simulink model "Inverter_pq_comp_sat"  (R2023b)
settings: Solver=FixedStepDiscrete  StartTime=0.0  StopTime=0.04  RelTol=1e-3  EnableMultiTasking=on
InitFcn:
  | %% Definition of the parameters
  | 
  | Parameter_Definition
  | 
  | %% Damping
  | 
  | Rd = 3.9;
  | 
  | %% PRes Gains Calculation
  | 
  | % Definicao das grandezas
  | w_cl = 1j*2*pi*1200;  % Phase Crossing Frequency
  | no   = 1;           % Integral Resonant Constant
  | A    = 1;             % Carrier Amplitude
  | 
  | % Kp calculation
  | a0 = 1;
  | a1 = Rd*Cf;
  | b0 = 0;
  | b1 = Lf+Lg;
  | b2 = Rd*Lf*Cf+Rd*Lg*Cf;
  | b3 = Lf*Lg*Cf;
  | 
  | G_lcl = (a1*w_cl+a0)/(b3*w_cl^3+b2*w_cl^2+b1*w_cl+b0);
  | % G_lcl = 1/((Lf+Lg)*w_cl+Rf);
  | 
  | G_PWM = (1/A)*(1-w_cl*Ts/4)/(1+w_cl*Ts/4);
  | 
  | G_wc  = (Vdc/2)*(1/I_base)*G_lcl*G_PWM;
  | 
  | G_wc_abs = abs(G_wc);
  | 
  | Kp = 0.8/G_wc_abs;
  | 
  | % Discretized Controller Gains
  | ressonance_list = [1,5,7];
  | 
  | n_res = length(ressonance_list);
  | a = zeros(2,n_res);
  | b = zeros(2,n_res);
  | Ki_res = zeros(1,n_res);
  | 
  | % for i = 1:n_res
  | %   k = ressonance_list(i);
  | %   Ki_res(i) = (2.2*Kp)/(no*T_gr);
  | %   a(i) = (2*Ki_res(i)*Ts)/(4+((k*w_gr)^2)*Ts^2);
  | %   b(i) = (-8+2*((k*w_gr)^2)*Ts^2)/(4+((k*w_gr)^2)*Ts^2);
  | % end
  | 
  | % wc is the cutoff frequency/damping factor in rad/s
  | wc = 5;
  | 
  | for i = 1:n_res
  |   k = ressonance_list(i);
  |   wk = k * w_gr; % Resonant frequency for this harmonic
  | 
  |   Ki_res(i) = (2.2*Kp)/(no*T_gr);
  | 
  |   % 1. Calculate the common denominator
  |   den = 4 + 4*wc*Ts + (wk^2)*(Ts^2);
  | 
  |   % 2. Calculate the numerator terms (A coefficients for the input x)
  |   num_A0 = 2 * Ki_res(i) * wc * Ts;
  | 
  |   % 3. Calculate the denominator terms (B coefficients for the output y)
  |   num_B1 = -8 + 2*(wk^2)*(Ts^2);
  |   num_B2 = 4 - 4*wc*Ts + (wk^2)*(Ts^2);
  | 
  |   % 4. Normalize the coefficients
  |   a(1,i) = num_A0 / den;
  |   a(2,i) = -1*num_A0 / den;
  |   b(1,i) = num_B1 / den;
  |   b(2,i) = num_B2 / den;
  | end
values from neighbouring files (symbols this model uses):
  a1_sogi = single(2*(w0_sogi^2-c_sogi^2)/den0_sogi)    [Parameter_Definition.m]
  a2_sogi = single((c_sogi^2                 - k_sogi*w0_sogi*c_sogi                 + w0_sogi^2)/den0_sogi)    [Parameter_Definition.m]
  bD_sogi = single(k_sogi*w0_sogi*c_sogi/den0_sogi)    [Parameter_Definition.m]
  bQ_sogi = single(k_sogi*w0_sogi^2/den0_sogi)    [Parameter_Definition.m]
  Cf = 5e-6    (= 5e-06)    [Parameter_Definition.m]
  I_base = S_base/(sqrt(3)*V_gr)    [Parameter_Definition.m]
  K_i = 1/25    (= 0.04)    [Parameter_Definition.m]
  K_vc = 1/200    (= 0.005)    [Parameter_Definition.m]
  K_vdc = 1/500    (= 0.002)    [Parameter_Definition.m]
  Lf = 1e-3    (= 0.001)    [Parameter_Definition.m]
  Lg = 0.5e-3    (= 0.0005)    [Parameter_Definition.m]
  S_base = S_rated    (= 1000)    [Parameter_Definition.m]
  Ts = 2*(4167)/100e6    (= 8.334e-05)    [Parameter_Definition.m]
  V_base = sqrt(3)*V_gr    [Parameter_Definition.m]
  Vdc = 800    [Parameter_Definition.m]
  Vdc_base = Vdc    (= 800)    [Parameter_Definition.m]
  w_gr = 2*pi*f_gr    (= 376.991118431)    [Parameter_Definition.m]
undefined symbols (not defined in the file or in its folder): Down, gH_LUT, GPTRIP1SEL, gQ_LUT, gV_LUT, lH_vetor, lQ_vetor, lV_vetor, TZ1, Up
libraries: c2802xlib x32, c2837xDlib x4, simulink x1
(part 1 of 3)
settings Model: SimulationMode=external  ExtModeTrigDuration=8  Creator=AugustoMatheusdosSan  LastModifiedBy=engam
settings SolverCC: AutoInsertRateTranBlk=on
settings OptimizationCC: DefaultUnderspecifiedDataType=single  EnhancedBackFolding=on  PassReuseOutputArgsAs=Individual arguments  MaxStackSize=1024  OptimizeBlockOrder=speed  DifferentSizesBufferReuse=on  OptimizationCustomize=off  EfficientTunableParamExpr=on
settings DebuggingCC: ParameterPrecisionLossMsg=none  ParameterTunabilityLossMsg=error
settings HardwareCC: ProdBitPerChar=16  ProdBitPerInt=16  ProdBitPerPointer=32  ProdBitPerSizeT=32  ProdBitPerPtrDiffT=32  ProdLargestAtomicInteger=Integer  ProdLargestAtomicFloat=None  ProdWordSize=16  ProdLongLongMode=on  ProdHWDeviceType=Texas Instruments->C2000  HardwareBoardFeatureSet=SoCBlockset
settings ModelReferenceCC: ModelReferenceNumInstancesAllowed=Single
settings SFSimCC: MATLABDynamicMemAlloc=off
settings RTWCC: Description=Embedded Coder  SystemTargetFile=ert.tlc  HardwareBoard=TI Delfino F2837xD  TemplateMakefile=ert_default_tmf  Toolchain=Texas Instruments Code Composer Studio (C2000)  BuildConfiguration=Faster Runs  CodeProfilingSaveOptions=MetricsOnly
settings CodeAppCC: ForceParamTrailComments=on  IgnoreCustomStorageClasses=off  OperatorAnnotations=on  SimulinkDataObjDesc=on  SFDataObjDesc=on  InsertBlockDesc=on
settings ERTTargetCC: TargetLangStandard=C99 (ISO)  CodeReplacementLibrary=TI C28x  ExtModeTransport=4  ExtModeStaticAlloc=on  ExtModeAutomaticAllocSize=off  ExtModeStaticAllocSize=10000  ExtModeMexFile=ext_xcp  ExtModeIntrfLevel=Level2 - Open  EnableUserReplacementTypes=on

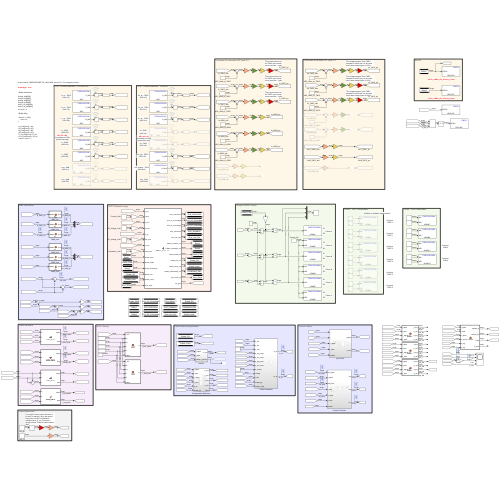
[thumbnail: Simulink's stored preview of the top-level diagram]
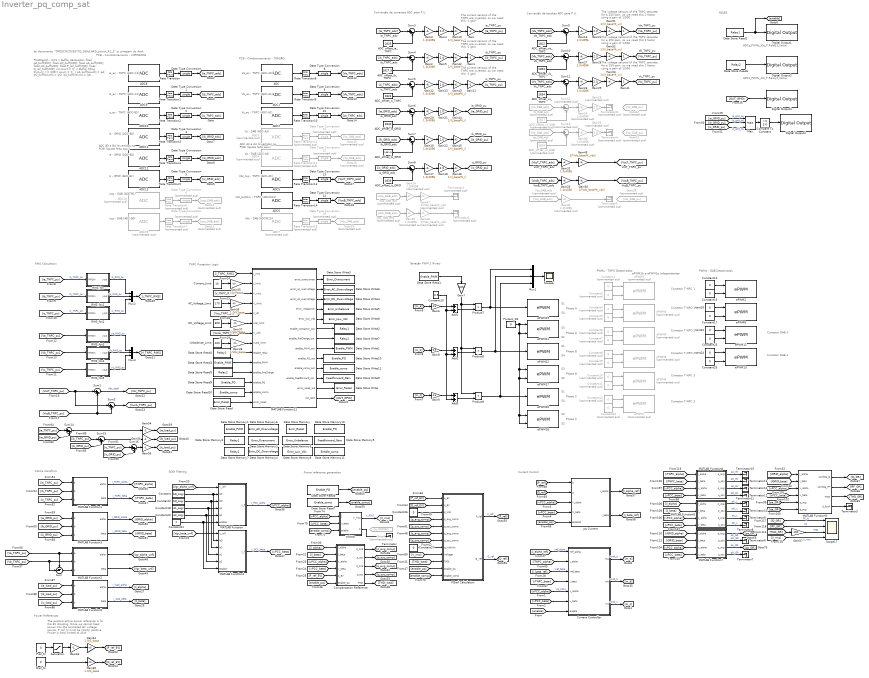
== system Inverter_pq_comp_sat ==
  note: S1
  note: Phase C
  note: The current sensors of the TNPC are inverted, so we need this -1 gain
  note: Conector
      | DAB 3
  note: Conversão de tensões ADC para P.U.
  note: S4
  note: Geração PWM 2 Níveis
  note: Phase C
  note: The current sensors of the TNPC are inverted, so we need this -1 gain
  note: RELÉS
  note: PlotGrapgh - CCS
      |
      | // Buffer declaration
      |
      | float pA_buff[200];
      | float pO_buff[200];
      | float qA_buff[200];
      | float qO_buff[200];
      | float P_ref_buff[200];
      | float Q_ref_buff[200];
      | int count = 0;
      |
      | // Buffer filling
      |
      | if(count >= 200){
      | count = 0;
      | }
      |
      | pA_buff[count] = pA;
      | pO_buff[count] = pO;
      | qA_buff[count] = qA;
      | qO_buff[count] = qO;
      | P_ref_buff[count] = P_ref;
      | Q_ref_buff[count] = Q_ref;
      | count = count + 1;
  note: PWMs - TNPC Desativados
  note: Conversão de correntes ADC para P.U.
  note: ib_ac - TNPC
      | (ADC-C2)
  note: ler documento "TMDSCNCD28377D_180cCARD_pinout_R1_3" p/ pinagem do dock
  note: Vp - DAB
      | (ADC-A4)
  note: PCB - Condicionamento - CORRENTE
  note: Vdc_bottom - TNPC
      | (ADCIN14)
  note: Vb_ac - TNPC
      | (ADC-A1)
  note: Va_ac - TNPC
      | (ADC-A0)
  note: The current sensors of the TNPC are inverted, so we need this -1 gain
  note: Vdc_top - TNPC
      | (ADC-A5)
  note: Vdc - DAB
      | (ADCIN15)
  note: Vs - DAB
      | (ADC-A3)
  note: ic_ac - TNPC
      | (ADC-B5)
  note: ia_ac - TNPC
      | (ADC-C3)
  note: ib - GRID
      | (ADC-B4)
  note: ia - GRID
      | (ADC-B3)
  note: S2
  note: ADCs_PWMs_IOs_P.Relay2_Value
  note: PWMs - DAB Desativados
  note: ADCs_PWMs_IOs_P.Relay1_Value
  note: iccp - DAB
      | (ADC-B1)
  note: iccs - DAB
      | (ADC-B0)
  note: ADC A3 e A4
      | (Invertidos na PCB)
      | (Ajuste feito aqui)
  note: Conector
      | T-NPC 1
  note: ADC B3 e B4
      | (Invertidos na PCB)
      | (Ajuste feito aqui)
  note: Conector
      | T-NPC 2
  note: ePWM1b e ePWM1a independentes
  note: ic - GRID
      | (ADC-B2)
  note: Conector
      | DAB 4
  note: Conector
      | T-NPC 2
  note: Conector
      | T-NPC 3
  note: Phase A
  note: S1
  note: S2
  note: S3
  note: Phase A
  note: PCB - Condicionamento - TENSÃO
  note: S1
  note: Conector
      | T-NPC 1
  note: S4
  note: S2
  note: S3
  note: Phase B
  note: S3
  note: Conector
      | T-NPC 3
  note: Phase B
  note: Vc_ac - TNPC
      | (ADC-A2)
  note: S4
  note: The voltage sensors of the TNPC saturate for a 250 gain, so we need this 2 factor using a gain of 1/500
  note: The voltage sensors of the TNPC saturate for a 250 gain, so we need this 2 factor using a gain of 1/500
  note: The voltage sensors of the TNPC saturate for a 250 gain, so we need this 2 factor using a gain of 1/500
  note: RMS Calculation
  note: The positive active power reference is for the EV charging. Since we cannot feed power into the controlled AC voltage source, P_ref_SI must be strictly positive. Power is hard limited to 4kW
  note: Power References
  note: TNPC Protection Logic
  note: SOGI Filtering
  note: Clarke transform
  note: Current Control
  note: Power reference generation
  AC_Voltage_Limit : Constant  Value=170  OutDataTypeStr=single
  ADC : c2802xlib/ADC  blkParamProc=C2000_Type4  ADCModule=A  samplingMode=Single sample mode  ADCResolution=12-bit (Single-ended input)  useSOC1=SOC0  useSOC2=SOC0_SOC1  SOCAcquisitionWindow=15  SOCTriggerSource=ePWM1_ADCSOCA  SOCInterruptTrigger=No ADCINT  Ts=Ts  dType=single  postInterrupt=off  interruptSel=ADCINT1  ADCINTContinuous=on  endma=off  chdma=1  conv1=ADCINA0  conv2=ADCINA0 and ADCINB0  conv1_Type4=ADCIN0  conv2_Type4=ADCIN0 and ADCIN1
      settings: LibrarySourceBlock=c2837xDlib/ADC
  ADC1 : c2802xlib/ADC  blkParamProc=C2000_Type4  ADCModule=A  samplingMode=Single sample mode  ADCResolution=12-bit (Single-ended input)  useSOC1=SOC1  useSOC2=SOC0_SOC1  SOCAcquisitionWindow=15  SOCTriggerSource=ePWM1_ADCSOCA  SOCInterruptTrigger=No ADCINT  Ts=Ts  dType=single  postInterrupt=off  interruptSel=ADCINT1  ADCINTContinuous=on  endma=off  chdma=1  conv1=ADCINA0  conv2=ADCINA0 and ADCINB0  conv1_Type4=ADCIN1  conv2_Type4=ADCIN0 and ADCIN1
      settings: LibrarySourceBlock=c2837xDlib/ADC
  ADC10 : c2802xlib/ADC  blkParamProc=C2000_Type4  ADCModule=B  samplingMode=Single sample mode  ADCResolution=12-bit (Single-ended input)  useSOC1=SOC10  useSOC2=SOC0_SOC1  SOCAcquisitionWindow=15  SOCTriggerSource=ePWM1_ADCSOCA  SOCInterruptTrigger=No ADCINT  Ts=Ts  dType=single  postInterrupt=off  interruptSel=ADCINT1  ADCINTContinuous=on  endma=off  chdma=1  conv1=ADCINA0  conv2=ADCINA0 and ADCINB0  conv1_Type4=ADCIN5  conv2_Type4=ADCIN0 and ADCIN1
      settings: LibrarySourceBlock=c2837xDlib/ADC
  ADC11 : c2802xlib/ADC  blkParamProc=C2000_Type4  ADCModule=B  samplingMode=Single sample mode  ADCResolution=12-bit (Single-ended input)  useSOC1=SOC11  useSOC2=SOC0_SOC1  SOCAcquisitionWindow=15  SOCTriggerSource=ePWM1_ADCSOCA  SOCInterruptTrigger=No ADCINT  Ts=Ts  dType=double  postInterrupt=off  interruptSel=ADCINT1  ADCINTContinuous=on  endma=off  chdma=1  conv1=ADCINA0  conv2=ADCINA0 and ADCINB0  conv1_Type4=ADCIN4  conv2_Type4=ADCIN0 and ADCIN1
      settings: LibrarySourceBlock=c2837xDlib/ADC
  ADC12 : c2802xlib/ADC  blkParamProc=C2000_Type4  ADCModule=B  samplingMode=Single sample mode  ADCResolution=12-bit (Single-ended input)  useSOC1=SOC12  useSOC2=SOC0_SOC1  SOCAcquisitionWindow=15  SOCTriggerSource=ePWM1_ADCSOCA  SOCInterruptTrigger=No ADCINT  Ts=Ts  dType=double  postInterrupt=off  interruptSel=ADCINT1  ADCINTContinuous=on  endma=off  chdma=1  conv1=ADCINA0  conv2=ADCINA0 and ADCINB0  conv1_Type4=ADCIN3  conv2_Type4=ADCIN0 and ADCIN1
      settings: LibrarySourceBlock=c2837xDlib/ADC
  ADC13 : c2802xlib/ADC  blkParamProc=C2000_Type4  ADCModule=B  samplingMode=Single sample mode  ADCResolution=12-bit (Single-ended input)  useSOC1=SOC13  useSOC2=SOC0_SOC1  SOCAcquisitionWindow=15  SOCTriggerSource=ePWM1_ADCSOCA  SOCInterruptTrigger=No ADCINT  Ts=Ts  dType=double  postInterrupt=off  interruptSel=ADCINT1  ADCINTContinuous=on  endma=off  chdma=1  conv1=ADCINA0  conv2=ADCINA0 and ADCINB0  conv1_Type4=ADCIN2  conv2_Type4=ADCIN0 and ADCIN1
      settings: LibrarySourceBlock=c2837xDlib/ADC
  ADC14 : c2802xlib/ADC  Commented=on  blkParamProc=C2000_Type4  ADCModule=B  samplingMode=Single sample mode  ADCResolution=12-bit (Single-ended input)  useSOC1=SOC14  useSOC2=SOC0_SOC1  SOCAcquisitionWindow=15  SOCTriggerSource=Software  SOCInterruptTrigger=No ADCINT  Ts=Ts  dType=double  postInterrupt=off  interruptSel=ADCINT1  ADCINTContinuous=on  endma=off  chdma=1  conv1=ADCINA0  conv2=ADCINA0 and ADCINB0  conv1_Type4=ADCIN1  conv2_Type4=ADCIN0 and ADCIN1
      settings: LibrarySourceBlock=c2837xDlib/ADC
  ADC15 : c2802xlib/ADC  Commented=on  blkParamProc=C2000_Type4  ADCModule=B  samplingMode=Single sample mode  ADCResolution=12-bit (Single-ended input)  useSOC1=SOC15  useSOC2=SOC0_SOC1  SOCAcquisitionWindow=15  SOCTriggerSource=Software  SOCInterruptTrigger=No ADCINT  Ts=Ts  dType=double  postInterrupt=off  interruptSel=ADCINT1  ADCINTContinuous=on  endma=off  chdma=1  conv1=ADCINA0  conv2=ADCINA0 and ADCINB0  conv1_Type4=ADCIN0  conv2_Type4=ADCIN0 and ADCIN1
      settings: LibrarySourceBlock=c2837xDlib/ADC
  ADC2 : c2802xlib/ADC  blkParamProc=C2000_Type4  ADCModule=A  samplingMode=Single sample mode  ADCResolution=12-bit (Single-ended input)  useSOC1=SOC2  useSOC2=SOC0_SOC1  SOCAcquisitionWindow=15  SOCTriggerSource=ePWM1_ADCSOCA  SOCInterruptTrigger=No ADCINT  Ts=Ts  dType=double  postInterrupt=off  interruptSel=ADCINT1  ADCINTContinuous=on  endma=off  chdma=1  conv1=ADCINA0  conv2=ADCINA0 and ADCINB0  conv1_Type4=ADCIN2  conv2_Type4=ADCIN0 and ADCIN1
      settings: LibrarySourceBlock=c2837xDlib/ADC
  ADC3 : c2802xlib/ADC  Commented=on  blkParamProc=C2000_Type4  ADCModule=A  samplingMode=Single sample mode  ADCResolution=12-bit (Single-ended input)  useSOC1=SOC3  useSOC2=SOC0_SOC1  SOCAcquisitionWindow=15  SOCTriggerSource=Software  SOCInterruptTrigger=No ADCINT  Ts=Ts  dType=double  postInterrupt=off  interruptSel=ADCINT1  ADCINTContinuous=on  endma=off  chdma=1  conv1=ADCINA0  conv2=ADCINA0 and ADCINB0  conv1_Type4=ADCIN3  conv2_Type4=ADCIN0 and ADCIN1
      settings: LibrarySourceBlock=c2837xDlib/ADC
  ADC4 : c2802xlib/ADC  Commented=on  blkParamProc=C2000_Type4  ADCModule=A  samplingMode=Single sample mode  ADCResolution=12-bit (Single-ended input)  useSOC1=SOC4  useSOC2=SOC0_SOC1  SOCAcquisitionWindow=15  SOCTriggerSource=Software  SOCInterruptTrigger=No ADCINT  Ts=Ts  dType=double  postInterrupt=off  interruptSel=ADCINT1  ADCINTContinuous=on  endma=off  chdma=1  conv1=ADCINA0  conv2=ADCINA0 and ADCINB0  conv1_Type4=ADCIN4  conv2_Type4=ADCIN0 and ADCIN1
      settings: LibrarySourceBlock=c2837xDlib/ADC
  ADC5 : c2802xlib/ADC  blkParamProc=C2000_Type4  ADCModule=A  samplingMode=Single sample mode  ADCResolution=12-bit (Single-ended input)  useSOC1=SOC5  useSOC2=SOC0_SOC1  SOCAcquisitionWindow=15  SOCTriggerSource=ePWM1_ADCSOCA  SOCInterruptTrigger=No ADCINT  Ts=Ts  dType=single  postInterrupt=off  interruptSel=ADCINT1  ADCINTContinuous=on  endma=off  chdma=1  conv1=ADCINA0  conv2=ADCINA0 and ADCINB0  conv1_Type4=ADCIN5  conv2_Type4=ADCIN0 and ADCIN1
      settings: LibrarySourceBlock=c2837xDlib/ADC
  ADC6 : c2802xlib/ADC  blkParamProc=C2000_Type4  ADCModule=A  samplingMode=Single sample mode  ADCResolution=12-bit (Single-ended input)  useSOC1=SOC6  useSOC2=SOC0_SOC1  SOCAcquisitionWindow=15  SOCTriggerSource=ePWM1_ADCSOCA  SOCInterruptTrigger=No ADCINT  Ts=Ts  dType=single  postInterrupt=on  interruptSel=ADCINT1  ADCINTContinuous=on  endma=off  chdma=1  conv1=ADCINA0  conv2=ADCINA0 and ADCINB0  conv1_Type4=ADCIN14  conv2_Type4=ADCIN0 and ADCIN1
      settings: LibrarySourceBlock=c2837xDlib/ADC
  ADC7 : c2802xlib/ADC  Commented=on  blkParamProc=C2000_Type4  ADCModule=A  samplingMode=Single sample mode  ADCResolution=12-bit (Single-ended input)  useSOC1=SOC7  useSOC2=SOC0_SOC1  SOCAcquisitionWindow=15  SOCTriggerSource=Software  SOCInterruptTrigger=No ADCINT  Ts=Ts  dType=double  postInterrupt=off  interruptSel=ADCINT1  ADCINTContinuous=on  endma=off  chdma=1  conv1=ADCINA0  conv2=ADCINA0 and ADCINB0  conv1_Type4=ADCIN15  conv2_Type4=ADCIN0 and ADCIN1
      settings: LibrarySourceBlock=c2837xDlib/ADC
  ADC8 : c2802xlib/ADC  blkParamProc=C2000_Type4  ADCModule=C  samplingMode=Single sample mode  ADCResolution=12-bit (Single-ended input)  useSOC1=SOC8  useSOC2=SOC0_SOC1  SOCAcquisitionWindow=15  SOCTriggerSource=ePWM1_ADCSOCA  SOCInterruptTrigger=No ADCINT  Ts=Ts  dType=single  postInterrupt=off  interruptSel=ADCINT1  ADCINTContinuous=on  endma=off  chdma=1  conv1=ADCINA0  conv2=ADCINA0 and ADCINB0  conv1_Type4=ADCIN3  conv2_Type4=ADCIN0 and ADCIN1
      settings: LibrarySourceBlock=c2837xDlib/ADC
  ADC9 : c2802xlib/ADC  blkParamProc=C2000_Type4  ADCModule=C  samplingMode=Single sample mode  ADCResolution=12-bit (Single-ended input)  useSOC1=SOC9  useSOC2=SOC0_SOC1  SOCAcquisitionWindow=15  SOCTriggerSource=ePWM1_ADCSOCA  SOCInterruptTrigger=No ADCINT  Ts=Ts  dType=single  postInterrupt=off  interruptSel=ADCINT1  ADCINTContinuous=on  endma=off  chdma=1  conv1=ADCINA0  conv2=ADCINA0 and ADCINB0  conv1_Type4=ADCIN2  conv2_Type4=ADCIN0 and ADCIN1
      settings: LibrarySourceBlock=c2837xDlib/ADC
  ADC_offset_ia_GRID : Constant  Value=1840  OutDataTypeStr=single
  ADC_offset_ia_TNPC : Constant  Value=1825  OutDataTypeStr=single
  ADC_offset_ib_GRID : Constant  Value=1831.5  OutDataTypeStr=single
  ADC_offset_ib_TNPC : Constant  Value=1827.5  OutDataTypeStr=single
  ADC_offset_ic_GRID : Constant  Value=1839  OutDataTypeStr=single
  ADC_offset_ic_TNPC : Constant  Value=1823  OutDataTypeStr=single
  ADC_offset_va_TNPC : Constant  Value=1822  OutDataTypeStr=single
  ADC_offset_vb_TNPC : Constant  Value=1853  OutDataTypeStr=single
  ADC_offset_vc_TNPC : Constant  Value=1834  OutDataTypeStr=single
  ADC_offset_vp_DAB : Constant  Commented=on  Value=1824  OutDataTypeStr=single
  ADC_offset_vs_DAB : Constant  Commented=on  Value=1817  OutDataTypeStr=single
  Add1 : Sum
  Add2 : Sum
  Add5 : Sum
  Compare To Constant : simulink/Logic and Bit Operations/Compare To Constant  relop=<=  const=3.0  OutDataTypeStr=boolean
  Compensation Reference : Subsystem
  Constant : Constant  Value=bD_sogi
  Constant{1,3..13} (12 alike) : Constant  Commented=on  Value=0  SampleTime=1/(12e3)
  Constant{14..17,22..25} (8 alike) : Constant  Value=0  SampleTime=Ts
  Constant18 : Constant  Value=a1_sogi
  Constant19 : Constant  Value=0.5  OutDataTypeStr=single
  Constant2 : Constant  Value=bQ_sogi
  Constant20 : Constant  Value=a2_sogi
  Constant21 : Constant
  Constant26 : Constant  Value=0  OutDataTypeStr=single
  Constant27 : Constant  Value=0  OutDataTypeStr=single
  Current Controller : Subsystem
  Current_Limit : Constant  Value=15  OutDataTypeStr=single
  DC_Voltage_Limit : Constant  Value=600  OutDataTypeStr=single
  Data Store Memory : DataStoreMemory  DataStoreName=Error_Reset  WriteAfterWriteMsg=warning  ShowAdditionalParam=off  OutDataTypeStr=single
  Data Store Memory1 : DataStoreMemory  DataStoreName=Enable_PWM  WriteAfterWriteMsg=warning  ShowAdditionalParam=off  OutDataTypeStr=single
  Data Store Memory10 : DataStoreMemory  DataStoreName=Enable_PQ  WriteAfterWriteMsg=warning  ShowAdditionalParam=off  OutDataTypeStr=single
  Data Store Memory11 : DataStoreMemory  DataStoreName=Enable_comp  WriteAfterWriteMsg=warning  ShowAdditionalParam=off  OutDataTypeStr=single
  Data Store Memory2 : DataStoreMemory  DataStoreName=Relay1  WriteAfterWriteMsg=warning  ShowAdditionalParam=off  OutDataTypeStr=single
  Data Store Memory3 : DataStoreMemory  DataStoreName=Error_Overcurrent  WriteAfterWriteMsg=warning  ShowAdditionalParam=off  OutDataTypeStr=single
  Data Store Memory4 : DataStoreMemory  DataStoreName=Error_DC_Overvoltage  WriteAfterWriteMsg=warning  ShowAdditionalParam=off  OutDataTypeStr=single
  Data Store Memory5 : DataStoreMemory  DataStoreName=Error_Unbalance  WriteAfterWriteMsg=warning  ShowAdditionalParam=off  OutDataTypeStr=single
  Data Store Memory6 : DataStoreMemory  DataStoreName=Error_AC_Overvoltage  WriteAfterWriteMsg=warning  ShowAdditionalParam=off  OutDataTypeStr=single
  Data Store Memory7 : DataStoreMemory  DataStoreName=Relay2  WriteAfterWriteMsg=warning  ShowAdditionalParam=off  OutDataTypeStr=single
  Data Store Memory8 : DataStoreMemory  DataStoreName=Error_Low_Vdc  WriteAfterWriteMsg=warning  ShowAdditionalParam=off  OutDataTypeStr=single
  Data Store Memory9 : DataStoreMemory  DataStoreName=Feedforward_Gain  WriteAfterWriteMsg=warning  ShowAdditionalParam=off  OutDataTypeStr=single
  Data Store Read : DataStoreRead  DataStoreName=Error_Reset  SampleTime=Ts  IndexOptions=Index vector (dialog)  Indices=1  OutputSizes=1
  Data Store Read1 : DataStoreRead  DataStoreName=Enable_PWM  IndexOptions=Index vector (dialog)  Indices=1  OutputSizes=1
  Data Store Read10 : DataStoreRead  DataStoreName=Enable_comp  SampleTime=Ts  IndexOptions=Index vector (dialog)  Indices=1  OutputSizes=1
  Data Store Read2 : DataStoreRead  DataStoreName=Relay1  SampleTime=Ts  IndexOptions=Index vector (dialog)  Indices=1  OutputSizes=1
  Data Store Read3 : DataStoreRead  DataStoreName=Enable_PWM  SampleTime=Ts  IndexOptions=Index vector (dialog)  Indices=1  OutputSizes=1
  Data Store Read4 : DataStoreRead  DataStoreName=Relay1  SampleTime=Ts  IndexOptions=Index vector (dialog)  Indices=1  OutputSizes=1
  Data Store Read5 : DataStoreRead  DataStoreName=Relay2  SampleTime=Ts  IndexOptions=Index vector (dialog)  Indices=1  OutputSizes=1
  Data Store Read6 : DataStoreRead  DataStoreName=Relay2  SampleTime=Ts  IndexOptions=Index vector (dialog)  Indices=1  OutputSizes=1
  Data Store Read7 : DataStoreRead  DataStoreName=Enable_comp  SampleTime=Ts  IndexOptions=Index vector (dialog)  Indices=1  OutputSizes=1
  Data Store Read8 : DataStoreRead  DataStoreName=Enable_PQ  SampleTime=Ts  IndexOptions=Index vector (dialog)  Indices=1  OutputSizes=1
  Data Store Read9 : DataStoreRead  DataStoreName=Enable_PQ  SampleTime=Ts  IndexOptions=Index vector (dialog)  Indices=1  OutputSizes=1
  Data Store Write : DataStoreWrite  DataStoreName=Error_Reset  SampleTime=Ts  IndexOptions=Index vector (dialog)  Indices=1  OutputSizes=1
  Data Store Write1 : DataStoreWrite  DataStoreName=Enable_PWM  SampleTime=Ts  IndexOptions=Index vector (dialog)  Indices=1  OutputSizes=1
  Data Store Write10 : DataStoreWrite  DataStoreName=Enable_PQ  SampleTime=Ts  IndexOptions=Index vector (dialog)  Indices=1  OutputSizes=1
  Data Store Write11 : DataStoreWrite  DataStoreName=Enable_comp  SampleTime=Ts  IndexOptions=Index vector (dialog)  Indices=1  OutputSizes=1
  Data Store Write2 : DataStoreWrite  DataStoreName=Relay1  SampleTime=Ts  IndexOptions=Index vector (dialog)  Indices=1  OutputSizes=1
  Data Store Write3 : DataStoreWrite  DataStoreName=Error_Overcurrent  SampleTime=Ts  IndexOptions=Index vector (dialog)  Indices=1  OutputSizes=1
  Data Store Write4 : DataStoreWrite  DataStoreName=Error_DC_Overvoltage  SampleTime=Ts  IndexOptions=Index vector (dialog)  Indices=1  OutputSizes=1
  Data Store Write5 : DataStoreWrite  DataStoreName=Error_Unbalance  SampleTime=Ts  IndexOptions=Index vector (dialog)  Indices=1  OutputSizes=1
  Data Store Write6 : DataStoreWrite  DataStoreName=Error_AC_Overvoltage  SampleTime=Ts  IndexOptions=Index vector (dialog)  Indices=1  OutputSizes=1
  Data Store Write7 : DataStoreWrite  DataStoreName=Relay2  SampleTime=Ts  IndexOptions=Index vector (dialog)  Indices=1  OutputSizes=1
  Data Store Write8 : DataStoreWrite  DataStoreName=Error_Low_Vdc  SampleTime=Ts  IndexOptions=Index vector (dialog)  Indices=1  OutputSizes=1
  Data Store Write9 : DataStoreWrite  DataStoreName=Feedforward_Gain  SampleTime=Ts  IndexOptions=Index vector (dialog)  Indices=1  OutputSizes=1
  Data Type Conversion{,1..5,8..10,13..14} (11 alike) : DataTypeConversion  OutDataTypeStr=single  SaturateOnIntegerOverflow=off  RndMeth=Floor
  Data Type Conversion{6..7,11..12,15} (5 alike) : DataTypeConversion  Commented=on  OutDataTypeStr=single  SaturateOnIntegerOverflow=off  RndMeth=Floor
  Digital Output1 : c2837xDlib/Digital Output  GPIO_Number=GPIO32~GPIO39  GPIO_Bit0=off  GPIO_BIT0_Toggle=off  GPIO_Bit1=off  GPIO_BIT1_Toggle=off  GPIO_Bit2=off  GPIO_BIT2_Toggle=off  GPIO_Bit3=on  GPIO_BIT3_Toggle=off  GPIO_Bit4=off  GPIO_BIT4_Toggle=off  GPIO_Bit5=off  GPIO_BIT5_Toggle=off  GPIO_Bit6=off  GPIO_BIT6_Toggle=off  GPIO_Bit7=off  GPIO_BIT7_Toggle=off
  Digital Output2 : c2837xDlib/Digital Output  GPIO_Number=GPIO32~GPIO39  GPIO_Bit0=off  GPIO_BIT0_Toggle=off  GPIO_Bit1=off  GPIO_BIT1_Toggle=off  GPIO_Bit2=off  GPIO_BIT2_Toggle=off  GPIO_Bit3=off  GPIO_BIT3_Toggle=off  GPIO_Bit4=off  GPIO_BIT4_Toggle=off  GPIO_Bit5=on  GPIO_BIT5_Toggle=off  GPIO_Bit6=off  GPIO_BIT6_Toggle=off  GPIO_Bit7=off  GPIO_BIT7_Toggle=off
  Digital Output3 : c2837xDlib/Digital Output  GPIO_Number=GPIO64~GPIO71  GPIO_Bit0=off  GPIO_BIT0_Toggle=off  GPIO_Bit1=off  GPIO_BIT1_Toggle=off  GPIO_Bit2=off  GPIO_BIT2_Toggle=off  GPIO_Bit3=on  GPIO_BIT3_Toggle=off  GPIO_Bit4=off  GPIO_BIT4_Toggle=off  GPIO_Bit5=off  GPIO_BIT5_Toggle=off  GPIO_Bit6=off  GPIO_BIT6_Toggle=off  GPIO_Bit7=off  GPIO_BIT7_Toggle=off
  Digital Output4 : c2837xDlib/Digital Output  GPIO_Number=GPIO64~GPIO71  GPIO_Bit0=off  GPIO_BIT0_Toggle=off  GPIO_Bit1=off  GPIO_BIT1_Toggle=off  GPIO_Bit2=off  GPIO_BIT2_Toggle=off  GPIO_Bit3=off  GPIO_BIT3_Toggle=off  GPIO_Bit4=on  GPIO_BIT4_Toggle=off  GPIO_Bit5=off  GPIO_BIT5_Toggle=off  GPIO_Bit6=off  GPIO_BIT6_Toggle=off  GPIO_Bit7=off  GPIO_BIT7_Toggle=off
  Gain{,1,11,54..56,63} (7 alike) : Gain  Gain=-1
  Gain{10,42..46} (6 alike) : Gain  Gain=1/(I_base*K_i)
  Gain{2..3,12,16..17,19..20,26..27,32..33} (11 alike) : Gain  Gain=1.0/4096
  Gain{4..5,13,18,21..23,28..29} (9 alike) : Gain  Gain=2.0
  Gain{14..15,24,30,34} (5 alike) : Gain  Commented=on  Gain=1.0/4096
  Gain25 : Gain  Commented=on  Gain=2.0
  Gain31 : Gain  Commented=on  Gain=2.0
  Gain35 : Gain  Gain=1.0/I_base
  Gain36 : Gain  Gain=1.0/V_base
  Gain37 : Gain  Gain=1/Vdc_base
  Gain38 : Gain  Gain=1/Vdc_base
  Gain39 : Gain
  Gain40 : Gain
  Gain41 : Gain
  Gain47 : Gain  Commented=on  Gain=1/(Vdc_base*K_vdc)
  Gain48 : Gain  Commented=on  Gain=1/(Vdc_base*K_vdc)
  Gain49 : Gain  Gain=1/(Vdc_base*K_vdc)
  Gain50 : Gain  Gain=1/(Vdc_base*K_vdc)
  Gain51 : Gain  Gain=1/(V_base*K_vc)
  Gain52 : Gain  Gain=1/(V_base*K_vc)
  Gain53 : Gain  Gain=1/(V_base*K_vc)
  Gain57 : Gain  Gain=100
  Gain6 : Gain  Gain=0.5
  Gain64 : Gain  Gain=1.0/S_base
  Gain65 : Gain  Gain=1.0/S_base
  Gain7 : Gain  Gain=100
  Gain8 : Gain  Gain=0.5
  Gain9 : Gain  Gain=0.5
  Goto10 : Goto  Commented=on  GotoTag=iccp_DAB_adc
  Goto11 : Goto  Commented=on  GotoTag=iccs_DAB_adc
  Goto15 : Goto  Commented=on  GotoTag=Vs_DAB_adc
  Goto16 : Goto  Commented=on  GotoTag=Vp_DAB_adc
  Goto19 : Goto  Commented=on  GotoTag=Vcc_DAB_adc
  Goto24 : Goto  Commented=on  GotoTag=Vs_DAB_pu
  Goto25 : Goto  Commented=on  GotoTag=Vp_DAB_pu
  Goto26 : Goto  Commented=on  GotoTag=Vcc_DAB_pu
  Goto4 : Goto  Commented=on  GotoTag=q_VoltVAr
  MATLAB Function : MATLAB Function  TreatAsAtomicUnit=on
  MATLAB Function1 : MATLAB Function  TreatAsAtomicUnit=on
  MATLAB Function11 : MATLAB Function  TreatAsAtomicUnit=on
  MATLAB Function2 : MATLAB Function  TreatAsAtomicUnit=on
  MATLAB Function3 : MATLAB Function  TreatAsAtomicUnit=on
  MATLAB Function4 : MATLAB Function  TreatAsAtomicUnit=on
  MATLAB Function5 : MATLAB Function  TreatAsAtomicUnit=on
  MATLAB Function6 : MATLAB Function  TreatAsAtomicUnit=on
  MATLAB Function7 : MATLAB Function  TreatAsAtomicUnit=on
  MATLAB Function8 : MATLAB Function  TreatAsAtomicUnit=on
  MATLAB Function9 : MATLAB Function  TreatAsAtomicUnit=on
  Max : MinMax  Function=max  Inputs=3
  Mux1 : Mux  Inputs=3
  Mux2 : Mux  Inputs=3
  Mux3 : Mux  Inputs=3
  PQref Calculation : Subsystem
  Porcent_D4 : Constant  Value=0
  Pref_SI : Constant  Value=0  OutDataTypeStr=single
  Product7 : Product
  Product8 : Product
  Product9 : Product
  Qref_SI : Constant  Value=0  OutDataTypeStr=single
  RMS_fcn : MATLAB Function  TreatAsAtomicUnit=on
  RMS_fcn1 : MATLAB Function  TreatAsAtomicUnit=on
  RMS_fcn2 : MATLAB Function  TreatAsAtomicUnit=on
  RMS_fcn3 : MATLAB Function  TreatAsAtomicUnit=on
  RMS_fcn4 : MATLAB Function  TreatAsAtomicUnit=on
  RMS_fcn5 : MATLAB Function  TreatAsAtomicUnit=on
  Rate Transition : RateTransition  Deterministic=off  OutPortSampleTime=Ts
  Rate Transition{1..5,8..10,13..14} (10 alike) : RateTransition  OutPortSampleTime=Ts
  Rate Transition{6..7,11..12,15} (5 alike) : RateTransition  Commented=on  OutPortSampleTime=Ts
  Saturation : Saturate  UpperLimit=4000  LowerLimit=0
  Scope17 : Scope  NumInputPorts=4
  Scope6 : Scope
  Sum : Sum  Inputs=--|
  Sum{1,14..16} (4 alike) : Sum  Inputs=|++
  Sum{2..11} (10 alike) : Sum  Inputs=|+-
  Sum12 : Sum  Commented=on  Inputs=|+-
  Sum13 : Sum  Commented=on  Inputs=|+-
  Terminator{,3,6..15} (12 alike) : Terminator
  Terminator{1..2,4..5,21} (5 alike) : Terminator  Commented=on
  Unbalance_Limit : Constant  Value=100  OutDataTypeStr=single
  Vcc_DAB_adc : From  Commented=on  GotoTag=Vcc_DAB_adc
  VoltVAr : Subsystem
  Vp_DAB_adc : From  Commented=on  GotoTag=Vp_DAB_adc
  Vs_DAB_adc : From  Commented=on  GotoTag=Vs_DAB_adc
  ePWM1 : c2802xlib/ePWM  Commented=on  PwmType=C2000_Type4  useModule=ePWM1  ePWMxLINKTBPRD=Not Linked  periodUnits=Clock cycles  timerSource=Specify via dialog  timerPeriod_clk=4166  timerPeriod_sec=0.0001  tbshadow=Counter equals to zero  countingMode=Up-Down  phaseActiveEnable=Disable  phaseDirection=Count down after sync  phaseActive=0  synchronizationEnable=off  dcaevt1Sync=off  dcbevt1Sync=off  synchronizationOption=Disable  dcbevt1SyncOut=off  dcaevt1SyncOut=off  cmpdSyncOut=off  cmpcSyncOut=off  cmpbSyncOut=off  zeroSyncOut=off  swfSyncOut=off  perSynchronizationOption=Counter equals to period (CTR=PRD)  clockPrescale=1  HSclockPrescale=1  enswap=off  ePWMxAStatus=on  ePWMxAactionLogic1=Set  ePWMxAactionLogic2=Clear  ePWMxAactionLogic3=Clear  ePWMxAactionLogic4=Set  ePWMxAactionLogic5=Do nothing  ePWMxAactionLogic6=Do nothing  ePWMxACSFenable=off  ePWMxACSFvalue=Forcing disable  ePWMxASFreload=Zero  ePWMxBStatus=on  ePWMxBactionLogic1=Set  ePWMxBactionLogic2=Clear  ePWMxBactionLogic3=Do nothing  ePWMxBactionLogic4=Do nothing  ePWMxBactionLogic5=Clear  ePWMxBactionLogic6=Set  ePWMxBCSFenable=off  ePWMxBCSFvalue=Forcing disable  ePWMxBSFreload=Zero  ePWNxBOutWay=off  ePWMxLINKCMPA=Not Linked  CMPAUnits=Percentages  CMPASource=Input port  CMPAValue_per=50  CMPAValue_clk=32000  enCMPAshadow=Counter equals to zero (CTR=Zero)  ePWMxLINKCMPB=Not Linked  CMPBUnits=Percentages  CMPBSource=Input port  CMPBValue_per=50  CMPBValue_clk=32000  enCMPBshadow=Counter equals to zero (CTR=Zero)  ePWMxLINKCMPC=Not Linked  CMPCUnits=Clock cycles  CMPCSource=Specify via dialog  CMPCValue_per=50  CMPCValue_clk=32000  enCMPCshadow=Counter equals to zero (CTR=Zero)  ePWMxLINKCMPD=Not Linked  CMPDUnits=Clock cycles  CMPDSource=Specify via dialog  CMPDValue_per=50  CMPDValue_clk=32000  enCMPDshadow=Counter equals to zero (CTR=Zero)  enableDBePWMxA=off  enableDBePWMxB=off  enhalfcycle=off  DBpolarity=Active high (AH)  DBedgeDelay=Positive  DBSource_ePWMxA=ePWMxA  DBSource_ePWMxB=ePWMxA  DBPeriodUnits=Clock cycles  DBperiodSource=Specify via dialog  REDperiod=0  FEDperiod=0  REDperiod_sec=0  FEDperiod_sec=0  LoadModeDBRED=Immediate without using shadow  LoadModeDBFED=Immediate without using shadow  adcstartModuleA=on  adcrequestEventA=First event  adcstartEventA=Digital Compare Module A Event 1 start of conversion (DCAEVT1.soc)  adcstartEventA_type2=Counter equals to period (CTR=PRD)  adcstartModuleB=off  adcrequestEventB=First event  adcstartEventB=Counter equals to zero (CTR=Zero)  adcstartEventB_type2=Counter equals to zero (CTR=Zero)  intEn=off  intPrd=First event  intSel=Counter equals to zero (CTR=Zero)  intSel_type2=Counter equals to zero (CTR=Zero)  hrpe=off  enHRPWM=off  HRPWM_LoadMode=Counter equals to period (CTR=PRD)  HRPWM_CTLMode=Duty or Period control mode  HRPWM_EDGMode=Both edge  hrpeb=off  enHRPWMB=off  HRPWM_LoadModeB=Counter equals to zero (CTR=ZERO)  HRPWM_CTLModeB=Duty or Period control mode  HRPWM_EDGModeB=Both edge  enHRDBRED=off  enHRDBFED=off  enSFO=on  enautoconv=on  chopperEnable=off  chopperFrequency=1  chopperFirstwidth=1  chopperDuty=12.5%  tripZonesource=Specify via dialog  tzselOSHT1=off  tzselOSHT2=off  tzselOSHT3=off  tzselOSHDCAEV1=off  tzselOSHDCBEV1=off  tzselCBC1=off  tzselCBC2=off  tzselCBC3=off  tzselCBCDCAEV2=off  tzselCBCDCBEV2=off  tzselOSHT4=off  tzselOSHT5=off  tzselOSHT6=off  tzselCBC4=off  tzselCBC5=off  tzselCBC6=off  enTzOstIntr=off  enTzCbcIntr=off  enTzDCAEVT1Intr=off  enTzDCAEVT2Intr=off  enTzDCBEVT1Intr=off  enTzDCBEVT2Intr=off  ePWMxAforced=No action  ePWMxBforced=No action  DCAEVT1forced=No action  DCBEVT1forced=No action  DCAEVT2forced=No action  DCBEVT2forced=No action  dcah=Trip Zone 1 input (TZ1)  dcal=Trip Zone 2 input (TZ2)  dcbh=Trip Zone 1 input (TZ1)  dcbl=Trip Zone 2 input (TZ2)  dcah_type2=GPTRIP1SEL/(TZ1)  dcal_type2=GPTRIP1SEL/(TZ1)  dcbh_type2=GPTRIP1SEL/(TZ1)  dcbl_type2=GPTRIP1SEL/(TZ1)  gendcaevt1=Event disabled  gendcaevt2=Event disabled  gendcbevt1=Event disabled  gendcbevt2=Event disabled  dcaevt1src=DCAEVT1 with sync  dcaevt2src=DCAEVT2 with sync  dcbevt1src=DCBEVT1 with sync  dcbevt2src=DCBEVT2 with sync  pulsesel=Counter equals to zero (CTR=Zero)  blankinv=off  blankoffset=0  blankwidth=0  evsrcsel=Filtered version of DCAEVT1 (DCAEVT1FILT)  encape=off
      settings: LibrarySourceBlock=c2837xDlib/ePWM
  ePWM12 : c2802xlib/ePWM  PwmType=C2000_Type4  useModule=ePWM11  ePWMxLINKTBPRD=Not Linked  periodUnits=Clock cycles  timerSource=Specify via dialog  timerPeriod_clk=4167  timerPeriod_sec=0.0001  tbshadow=Counter equals to zero  countingMode=Up-Down  phaseActiveEnable=Disable  phaseDirection=Count down after sync  phaseActive=0  synchronizationEnable=off  dcaevt1Sync=off  dcbevt1Sync=off  synchronizationOption=Disable  dcbevt1SyncOut=off  dcaevt1SyncOut=off  cmpdSyncOut=off  cmpcSyncOut=off  cmpbSyncOut=off  zeroSyncOut=off  swfSyncOut=off  perSynchronizationOption=Counter equals to period (CTR=PRD)  clockPrescale=1  HSclockPrescale=1  enswap=off  ePWMxAStatus=on  ePWMxAactionLogic1=Set  ePWMxAactionLogic2=Clear  ePWMxAactionLogic3=Clear  ePWMxAactionLogic4=Set  ePWMxAactionLogic5=Do nothing  ePWMxAactionLogic6=Do nothing  ePWMxACSFenable=off  ePWMxACSFvalue=Forcing disable  ePWMxASFreload=Zero  ePWMxBStatus=on  ePWMxBactionLogic1=Set  ePWMxBactionLogic2=Clear  ePWMxBactionLogic3=Do nothing  ePWMxBactionLogic4=Do nothing  ePWMxBactionLogic5=Clear  ePWMxBactionLogic6=Set  ePWMxBCSFenable=off  ePWMxBCSFvalue=Forcing disable  ePWMxBSFreload=Zero  ePWNxBOutWay=off  ePWMxLINKCMPA=Not Linked  CMPAUnits=Percentages  CMPASource=Input port  CMPAValue_per=50  CMPAValue_clk=32000  enCMPAshadow=Counter equals to zero (CTR=Zero)  ePWMxLINKCMPB=Not Linked  CMPBUnits=Percentages  CMPBSource=Input port  CMPBValue_per=50  CMPBValue_clk=32000  enCMPBshadow=Counter equals to zero (CTR=Zero)  ePWMxLINKCMPC=Not Linked  CMPCUnits=Clock cycles  CMPCSource=Specify via dialog  CMPCValue_per=50  CMPCValue_clk=32000  enCMPCshadow=Counter equals to zero (CTR=Zero)  ePWMxLINKCMPD=Not Linked  CMPDUnits=Clock cycles  CMPDSource=Specify via dialog  CMPDValue_per=50  CMPDValue_clk=32000  enCMPDshadow=Counter equals to zero (CTR=Zero)  enableDBePWMxA=off  enableDBePWMxB=off  enhalfcycle=off  DBpolarity=Active high (AH)  DBedgeDelay=Positive  DBSource_ePWMxA=ePWMxA  DBSource_ePWMxB=ePWMxA  DBPeriodUnits=Clock cycles  DBperiodSource=Specify via dialog  REDperiod=0  FEDperiod=0  REDperiod_sec=0  FEDperiod_sec=0  LoadModeDBRED=Immediate without using shadow  LoadModeDBFED=Immediate without using shadow  adcstartModuleA=off  adcrequestEventA=First event  adcstartEventA=Digital Compare Module A Event 1 start of conversion (DCAEVT1.soc)  adcstartEventA_type2=Counter equals to zero (CTR=Zero)  adcstartModuleB=off  adcrequestEventB=First event  adcstartEventB=Counter equals to zero (CTR=Zero)  adcstartEventB_type2=Counter equals to zero (CTR=Zero)  intEn=off  intPrd=First event  intSel=Counter equals to zero (CTR=Zero)  intSel_type2=Counter equals to zero (CTR=Zero)  hrpe=off  enHRPWM=off  HRPWM_LoadMode=Counter equals to period (CTR=PRD)  HRPWM_CTLMode=Duty or Period control mode  HRPWM_EDGMode=Both edge  hrpeb=off  enHRPWMB=off  HRPWM_LoadModeB=Counter equals to zero (CTR=ZERO)  HRPWM_CTLModeB=Duty or Period control mode  HRPWM_EDGModeB=Both edge  enHRDBRED=off  enHRDBFED=off  enSFO=on  enautoconv=on  chopperEnable=off  chopperFrequency=1  chopperFirstwidth=1  chopperDuty=12.5%  tripZonesource=Specify via dialog  tzselOSHT1=off  tzselOSHT2=off  tzselOSHT3=off  tzselOSHDCAEV1=off  tzselOSHDCBEV1=off  tzselCBC1=off  tzselCBC2=off  tzselCBC3=off  tzselCBCDCAEV2=off  tzselCBCDCBEV2=off  tzselOSHT4=off  tzselOSHT5=off  tzselOSHT6=off  tzselCBC4=off  tzselCBC5=off  tzselCBC6=off  enTzOstIntr=off  enTzCbcIntr=off  enTzDCAEVT1Intr=off  enTzDCAEVT2Intr=off  enTzDCBEVT1Intr=off  enTzDCBEVT2Intr=off  ePWMxAforced=No action  ePWMxBforced=No action  DCAEVT1forced=No action  DCBEVT1forced=No action  DCAEVT2forced=No action  DCBEVT2forced=No action  dcah=Trip Zone 1 input (TZ1)  dcal=Trip Zone 2 input (TZ2)  dcbh=Trip Zone 1 input (TZ1)  dcbl=Trip Zone 2 input (TZ2)  dcah_type2=GPTRIP1SEL/(TZ1)  dcal_type2=GPTRIP1SEL/(TZ1)  dcbh_type2=GPTRIP1SEL/(TZ1)  dcbl_type2=GPTRIP1SEL/(TZ1)  gendcaevt1=Event disabled  gendcaevt2=Event disabled  gendcbevt1=Event disabled  gendcbevt2=Event disabled  dcaevt1src=DCAEVT1 with sync  dcaevt2src=DCAEVT2 with sync  dcbevt1src=DCBEVT1 with sync  dcbevt2src=DCBEVT2 with sync  pulsesel=Counter equals to zero (CTR=Zero)  blankinv=off  blankoffset=0  blankwidth=0  evsrcsel=Filtered version of DCAEVT1 (DCAEVT1FILT)  encape=off
      settings: LibrarySourceBlock=c2837xDlib/ePWM
  ePWM13 : c2802xlib/ePWM  PwmType=C2000_Type4  useModule=ePWM12  ePWMxLINKTBPRD=Not Linked  periodUnits=Clock cycles  timerSource=Specify via dialog  timerPeriod_clk=4167  timerPeriod_sec=0.0001  tbshadow=Counter equals to zero  countingMode=Up-Down  phaseActiveEnable=Disable  phaseDirection=Count down after sync  phaseActive=0  synchronizationEnable=off  dcaevt1Sync=off  dcbevt1Sync=off  synchronizationOption=Disable  dcbevt1SyncOut=off  dcaevt1SyncOut=off  cmpdSyncOut=off  cmpcSyncOut=off  cmpbSyncOut=off  zeroSyncOut=off  swfSyncOut=off  perSynchronizationOption=Counter equals to period (CTR=PRD)  clockPrescale=1  HSclockPrescale=1  enswap=off  ePWMxAStatus=on  ePWMxAactionLogic1=Set  ePWMxAactionLogic2=Clear  ePWMxAactionLogic3=Clear  ePWMxAactionLogic4=Set  ePWMxAactionLogic5=Do nothing  ePWMxAactionLogic6=Do nothing  ePWMxACSFenable=off  ePWMxACSFvalue=Forcing disable  ePWMxASFreload=Zero  ePWMxBStatus=on  ePWMxBactionLogic1=Set  ePWMxBactionLogic2=Clear  ePWMxBactionLogic3=Do nothing  ePWMxBactionLogic4=Do nothing  ePWMxBactionLogic5=Clear  ePWMxBactionLogic6=Set  ePWMxBCSFenable=off  ePWMxBCSFvalue=Forcing disable  ePWMxBSFreload=Zero  ePWNxBOutWay=off  ePWMxLINKCMPA=Not Linked  CMPAUnits=Percentages  CMPASource=Input port  CMPAValue_per=50  CMPAValue_clk=32000  enCMPAshadow=Counter equals to zero (CTR=Zero)  ePWMxLINKCMPB=Not Linked  CMPBUnits=Percentages  CMPBSource=Input port  CMPBValue_per=50  CMPBValue_clk=32000  enCMPBshadow=Counter equals to zero (CTR=Zero)  ePWMxLINKCMPC=Not Linked  CMPCUnits=Clock cycles  CMPCSource=Specify via dialog  CMPCValue_per=50  CMPCValue_clk=32000  enCMPCshadow=Counter equals to zero (CTR=Zero)  ePWMxLINKCMPD=Not Linked  CMPDUnits=Clock cycles  CMPDSource=Specify via dialog  CMPDValue_per=50  CMPDValue_clk=32000  enCMPDshadow=Counter equals to zero (CTR=Zero)  enableDBePWMxA=off  enableDBePWMxB=off  enhalfcycle=off  DBpolarity=Active high (AH)  DBedgeDelay=Positive  DBSource_ePWMxA=ePWMxA  DBSource_ePWMxB=ePWMxA  DBPeriodUnits=Clock cycles  DBperiodSource=Specify via dialog  REDperiod=0  FEDperiod=0  REDperiod_sec=0  FEDperiod_sec=0  LoadModeDBRED=Immediate without using shadow  LoadModeDBFED=Immediate without using shadow  adcstartModuleA=off  adcrequestEventA=First event  adcstartEventA=Digital Compare Module A Event 1 start of conversion (DCAEVT1.soc)  adcstartEventA_type2=Counter equals to zero (CTR=Zero)  adcstartModuleB=off  adcrequestEventB=First event  adcstartEventB=Counter equals to zero (CTR=Zero)  adcstartEventB_type2=Counter equals to zero (CTR=Zero)  intEn=off  intPrd=First event  intSel=Counter equals to zero (CTR=Zero)  intSel_type2=Counter equals to zero (CTR=Zero)  hrpe=off  enHRPWM=off  HRPWM_LoadMode=Counter equals to period (CTR=PRD)  HRPWM_CTLMode=Duty or Period control mode  HRPWM_EDGMode=Both edge  hrpeb=off  enHRPWMB=off  HRPWM_LoadModeB=Counter equals to zero (CTR=ZERO)  HRPWM_CTLModeB=Duty or Period control mode  HRPWM_EDGModeB=Both edge  enHRDBRED=off  enHRDBFED=off  enSFO=on  enautoconv=on  chopperEnable=off  chopperFrequency=1  chopperFirstwidth=1  chopperDuty=12.5%  tripZonesource=Specify via dialog  tzselOSHT1=off  tzselOSHT2=off  tzselOSHT3=off  tzselOSHDCAEV1=off  tzselOSHDCBEV1=off  tzselCBC1=off  tzselCBC2=off  tzselCBC3=off  tzselCBCDCAEV2=off  tzselCBCDCBEV2=off  tzselOSHT4=off  tzselOSHT5=off  tzselOSHT6=off  tzselCBC4=off  tzselCBC5=off  tzselCBC6=off  enTzOstIntr=off  enTzCbcIntr=off  enTzDCAEVT1Intr=off  enTzDCAEVT2Intr=off  enTzDCBEVT1Intr=off  enTzDCBEVT2Intr=off  ePWMxAforced=No action  ePWMxBforced=No action  DCAEVT1forced=No action  DCBEVT1forced=No action  DCAEVT2forced=No action  DCBEVT2forced=No action  dcah=Trip Zone 1 input (TZ1)  dcal=Trip Zone 2 input (TZ2)  dcbh=Trip Zone 1 input (TZ1)  dcbl=Trip Zone 2 input (TZ2)  dcah_type2=GPTRIP1SEL/(TZ1)  dcal_type2=GPTRIP1SEL/(TZ1)  dcbh_type2=GPTRIP1SEL/(TZ1)  dcbl_type2=GPTRIP1SEL/(TZ1)  gendcaevt1=Event disabled  gendcaevt2=Event disabled  gendcbevt1=Event disabled  gendcbevt2=Event disabled  dcaevt1src=DCAEVT1 with sync  dcaevt2src=DCAEVT2 with sync  dcbevt1src=DCBEVT1 with sync  dcbevt2src=DCBEVT2 with sync  pulsesel=Counter equals to zero (CTR=Zero)  blankinv=off  blankoffset=0  blankwidth=0  evsrcsel=Filtered version of DCAEVT1 (DCAEVT1FILT)  encape=off
      settings: LibrarySourceBlock=c2837xDlib/ePWM
  ePWM17 : c2802xlib/ePWM  PwmType=C2000_Type4  useModule=ePWM4  ePWMxLINKTBPRD=Not Linked  periodUnits=Clock cycles  timerSource=Specify via dialog  timerPeriod_clk=4167  timerPeriod_sec=0.0001  tbshadow=Counter equals to zero  countingMode=Up-Down  phaseActiveEnable=Disable  phaseDirection=Count down after sync  phaseActive=0  synchronizationEnable=off  dcaevt1Sync=off  dcbevt1Sync=off  synchronizationOption=Counter equals to zero (CTR=Zero)  dcbevt1SyncOut=off  dcaevt1SyncOut=off  cmpdSyncOut=off  cmpcSyncOut=off  cmpbSyncOut=off  zeroSyncOut=off  swfSyncOut=off  perSynchronizationOption=Counter equals to period (CTR=PRD)  clockPrescale=1  HSclockPrescale=1  enswap=off  ePWMxAStatus=on  ePWMxAactionLogic1=Set  ePWMxAactionLogic2=Clear  ePWMxAactionLogic3=Clear  ePWMxAactionLogic4=Set  ePWMxAactionLogic5=Do nothing  ePWMxAactionLogic6=Do nothing  ePWMxACSFenable=off  ePWMxACSFvalue=Forcing disable  ePWMxASFreload=Zero  ePWMxBStatus=on  ePWMxBactionLogic1=Set  ePWMxBactionLogic2=Clear  ePWMxBactionLogic3=Do nothing  ePWMxBactionLogic4=Do nothing  ePWMxBactionLogic5=Clear  ePWMxBactionLogic6=Set  ePWMxBCSFenable=off  ePWMxBCSFvalue=Forcing disable  ePWMxBSFreload=Zero  ePWNxBOutWay=off  ePWMxLINKCMPA=Not Linked  CMPAUnits=Percentages  CMPASource=Input port  CMPAValue_per=50  CMPAValue_clk=32000  enCMPAshadow=Counter equals to zero (CTR=Zero)  ePWMxLINKCMPB=Not Linked  CMPBUnits=Percentages  CMPBSource=Input port  CMPBValue_per=50  CMPBValue_clk=32000  enCMPBshadow=Counter equals to zero (CTR=Zero)  ePWMxLINKCMPC=Not Linked  CMPCUnits=Clock cycles  CMPCSource=Specify via dialog  CMPCValue_per=50  CMPCValue_clk=32000  enCMPCshadow=Counter equals to zero (CTR=Zero)  ePWMxLINKCMPD=Not Linked  CMPDUnits=Clock cycles  CMPDSource=Specify via dialog  CMPDValue_per=50  CMPDValue_clk=32000  enCMPDshadow=Counter equals to zero (CTR=Zero)  enableDBePWMxA=off  enableDBePWMxB=off  enhalfcycle=off  DBpolarity=Active high complementary (AHC)  DBedgeDelay=Positive  DBSource_ePWMxA=ePWMxA  DBSource_ePWMxB=ePWMxA  DBPeriodUnits=Clock cycles  DBperiodSource=Specify via dialog  REDperiod=200  FEDperiod=200  REDperiod_sec=0  FEDperiod_sec=0  LoadModeDBRED=Immediate without using shadow  LoadModeDBFED=Immediate without using shadow  adcstartModuleA=off  adcrequestEventA=First event  adcstartEventA=Digital Compare Module A Event 1 start of conversion (DCAEVT1.soc)  adcstartEventA_type2=Counter equals to zero (CTR=Zero)  adcstartModuleB=off  adcrequestEventB=First event  adcstartEventB=Counter equals to zero (CTR=Zero)  adcstartEventB_type2=Counter equals to zero (CTR=Zero)  intEn=off  intPrd=First event  intSel=Counter equals to zero (CTR=Zero)  intSel_type2=Counter equals to zero (CTR=Zero)  hrpe=off  enHRPWM=off  HRPWM_LoadMode=Counter equals to period (CTR=PRD)  HRPWM_CTLMode=Duty or Period control mode  HRPWM_EDGMode=Both edge  hrpeb=off  enHRPWMB=off  HRPWM_LoadModeB=Counter equals to zero (CTR=ZERO)  HRPWM_CTLModeB=Duty or Period control mode  HRPWM_EDGModeB=Both edge  enHRDBRED=off  enHRDBFED=off  enSFO=on  enautoconv=on  chopperEnable=off  chopperFrequency=1  chopperFirstwidth=1  chopperDuty=12.5%  tripZonesource=Specify via dialog  tzselOSHT1=off  tzselOSHT2=off  tzselOSHT3=off  tzselOSHDCAEV1=off  tzselOSHDCBEV1=off  tzselCBC1=off  tzselCBC2=off  tzselCBC3=off  tzselCBCDCAEV2=off  tzselCBCDCBEV2=off  tzselOSHT4=off  tzselOSHT5=off  tzselOSHT6=off  tzselCBC4=off  tzselCBC5=off  tzselCBC6=off  enTzOstIntr=off  enTzCbcIntr=off  enTzDCAEVT1Intr=off  enTzDCAEVT2Intr=off  enTzDCBEVT1Intr=off  enTzDCBEVT2Intr=off  ePWMxAforced=No action  ePWMxBforced=No action  DCAEVT1forced=No action  DCBEVT1forced=No action  DCAEVT2forced=No action  DCBEVT2forced=No action  dcah=Trip Zone 1 input (TZ1)  dcal=Trip Zone 2 input (TZ2)  dcbh=Trip Zone 1 input (TZ1)  dcbl=Trip Zone 2 input (TZ2)  dcah_type2=GPTRIP1SEL/(TZ1)  dcal_type2=GPTRIP1SEL/(TZ1)  dcbh_type2=GPTRIP1SEL/(TZ1)  dcbl_type2=GPTRIP1SEL/(TZ1)  gendcaevt1=Event disabled  gendcaevt2=Event disabled  gendcbevt1=Event disabled  gendcbevt2=Event disabled  dcaevt1src=DCAEVT1 with sync  dcaevt2src=DCAEVT2 with sync  dcbevt1src=DCBEVT1 with sync  dcbevt2src=DCBEVT2 with sync  pulsesel=Counter equals to zero (CTR=Zero)  blankinv=off  blankoffset=0  blankwidth=0  evsrcsel=Filtered version of DCAEVT1 (DCAEVT1FILT)  encape=off
      settings: LibrarySourceBlock=c2837xDlib/ePWM
  ePWM18 : c2802xlib/ePWM  PwmType=C2000_Type4  useModule=ePWM6  ePWMxLINKTBPRD=Not Linked  periodUnits=Clock cycles  timerSource=Specify via dialog  timerPeriod_clk=4167  timerPeriod_sec=0.0001  tbshadow=Counter equals to zero  countingMode=Up-Down  phaseActiveEnable=Disable  phaseDirection=Count down after sync  phaseActive=0  synchronizationEnable=off  dcaevt1Sync=off  dcbevt1Sync=off  synchronizationOption=Counter equals to zero (CTR=Zero)  dcbevt1SyncOut=off  dcaevt1SyncOut=off  cmpdSyncOut=off  cmpcSyncOut=off  cmpbSyncOut=off  zeroSyncOut=off  swfSyncOut=off  perSynchronizationOption=Counter equals to period (CTR=PRD)  clockPrescale=1  HSclockPrescale=1  enswap=off  ePWMxAStatus=on  ePWMxAactionLogic1=Set  ePWMxAactionLogic2=Clear  ePWMxAactionLogic3=Clear  ePWMxAactionLogic4=Set  ePWMxAactionLogic5=Do nothing  ePWMxAactionLogic6=Do nothing  ePWMxACSFenable=off  ePWMxACSFvalue=Forcing disable  ePWMxASFreload=Zero  ePWMxBStatus=on  ePWMxBactionLogic1=Set  ePWMxBactionLogic2=Clear  ePWMxBactionLogic3=Do nothing  ePWMxBactionLogic4=Do nothing  ePWMxBactionLogic5=Clear  ePWMxBactionLogic6=Set  ePWMxBCSFenable=off  ePWMxBCSFvalue=Forcing disable  ePWMxBSFreload=Zero  ePWNxBOutWay=off  ePWMxLINKCMPA=Not Linked  CMPAUnits=Percentages  CMPASource=Input port  CMPAValue_per=50  CMPAValue_clk=32000  enCMPAshadow=Counter equals to zero (CTR=Zero)  ePWMxLINKCMPB=Not Linked  CMPBUnits=Percentages  CMPBSource=Input port  CMPBValue_per=50  CMPBValue_clk=32000  enCMPBshadow=Counter equals to zero (CTR=Zero)  ePWMxLINKCMPC=Not Linked  CMPCUnits=Clock cycles  CMPCSource=Specify via dialog  CMPCValue_per=50  CMPCValue_clk=32000  enCMPCshadow=Counter equals to zero (CTR=Zero)  ePWMxLINKCMPD=Not Linked  CMPDUnits=Clock cycles  CMPDSource=Specify via dialog  CMPDValue_per=50  CMPDValue_clk=32000  enCMPDshadow=Counter equals to zero (CTR=Zero)  enableDBePWMxA=off  enableDBePWMxB=off  enhalfcycle=off  DBpolarity=Active high complementary (AHC)  DBedgeDelay=Positive  DBSource_ePWMxA=ePWMxA  DBSource_ePWMxB=ePWMxA  DBPeriodUnits=Clock cycles  DBperiodSource=Specify via dialog  REDperiod=200  FEDperiod=200  REDperiod_sec=0  FEDperiod_sec=0  LoadModeDBRED=Immediate without using shadow  LoadModeDBFED=Immediate without using shadow  adcstartModuleA=off  adcrequestEventA=First event  adcstartEventA=Digital Compare Module A Event 1 start of conversion (DCAEVT1.soc)  adcstartEventA_type2=Counter equals to zero (CTR=Zero)  adcstartModuleB=off  adcrequestEventB=First event  adcstartEventB=Counter equals to zero (CTR=Zero)  adcstartEventB_type2=Counter equals to zero (CTR=Zero)  intEn=off  intPrd=First event  intSel=Counter equals to zero (CTR=Zero)  intSel_type2=Counter equals to zero (CTR=Zero)  hrpe=off  enHRPWM=off  HRPWM_LoadMode=Counter equals to period (CTR=PRD)  HRPWM_CTLMode=Duty or Period control mode  HRPWM_EDGMode=Both edge  hrpeb=off  enHRPWMB=off  HRPWM_LoadModeB=Counter equals to zero (CTR=ZERO)  HRPWM_CTLModeB=Duty or Period control mode  HRPWM_EDGModeB=Both edge  enHRDBRED=off  enHRDBFED=off  enSFO=on  enautoconv=on  chopperEnable=off  chopperFrequency=1  chopperFirstwidth=1  chopperDuty=12.5%  tripZonesource=Specify via dialog  tzselOSHT1=off  tzselOSHT2=off  tzselOSHT3=off  tzselOSHDCAEV1=off  tzselOSHDCBEV1=off  tzselCBC1=off  tzselCBC2=off  tzselCBC3=off  tzselCBCDCAEV2=off  tzselCBCDCBEV2=off  tzselOSHT4=off  tzselOSHT5=off  tzselOSHT6=off  tzselCBC4=off  tzselCBC5=off  tzselCBC6=off  enTzOstIntr=off  enTzCbcIntr=off  enTzDCAEVT1Intr=off  enTzDCAEVT2Intr=off  enTzDCBEVT1Intr=off  enTzDCBEVT2Intr=off  ePWMxAforced=No action  ePWMxBforced=No action  DCAEVT1forced=No action  DCBEVT1forced=No action  DCAEVT2forced=No action  DCBEVT2forced=No action  dcah=Trip Zone 1 input (TZ1)  dcal=Trip Zone 2 input (TZ2)  dcbh=Trip Zone 1 input (TZ1)  dcbl=Trip Zone 2 input (TZ2)  dcah_type2=GPTRIP1SEL/(TZ1)  dcal_type2=GPTRIP1SEL/(TZ1)  dcbh_type2=GPTRIP1SEL/(TZ1)  dcbl_type2=GPTRIP1SEL/(TZ1)  gendcaevt1=Event disabled  gendcaevt2=Event disabled  gendcbevt1=Event disabled  gendcbevt2=Event disabled  dcaevt1src=DCAEVT1 with sync  dcaevt2src=DCAEVT2 with sync  dcbevt1src=DCBEVT1 with sync  dcbevt2src=DCBEVT2 with sync  pulsesel=Counter equals to zero (CTR=Zero)  blankinv=off  blankoffset=0  blankwidth=0  evsrcsel=Filtered version of DCAEVT1 (DCAEVT1FILT)  encape=off
      settings: LibrarySourceBlock=c2837xDlib/ePWM
  ePWM19 : c2802xlib/ePWM  PwmType=C2000_Type4  useModule=ePWM1  ePWMxLINKTBPRD=Not Linked  periodUnits=Clock cycles  timerSource=Specify via dialog  timerPeriod_clk=4167  timerPeriod_sec=0.0001  tbshadow=Counter equals to zero  countingMode=Up-Down  phaseActiveEnable=Disable  phaseDirection=Count down after sync  phaseActive=0  synchronizationEnable=off  dcaevt1Sync=off  dcbevt1Sync=off  synchronizationOption=Disable  dcbevt1SyncOut=off  dcaevt1SyncOut=off  cmpdSyncOut=off  cmpcSyncOut=off  cmpbSyncOut=off  zeroSyncOut=off  swfSyncOut=off  perSynchronizationOption=Counter equals to period (CTR=PRD)  clockPrescale=1  HSclockPrescale=1  enswap=off  ePWMxAStatus=on  ePWMxAactionLogic1=Set  ePWMxAactionLogic2=Clear  ePWMxAactionLogic3=Clear  ePWMxAactionLogic4=Set  ePWMxAactionLogic5=Do nothing  ePWMxAactionLogic6=Do nothing  ePWMxACSFenable=off  ePWMxACSFvalue=Forcing disable  ePWMxASFreload=Zero  ePWMxBStatus=on  ePWMxBactionLogic1=Set  ePWMxBactionLogic2=Clear  ePWMxBactionLogic3=Do nothing  ePWMxBactionLogic4=Do nothing  ePWMxBactionLogic5=Clear  ePWMxBactionLogic6=Set  ePWMxBCSFenable=off  ePWMxBCSFvalue=Forcing disable  ePWMxBSFreload=Zero  ePWNxBOutWay=off  ePWMxLINKCMPA=Not Linked  CMPAUnits=Percentages  CMPASource=Input port  CMPAValue_per=50  CMPAValue_clk=32000  enCMPAshadow=Counter equals to zero (CTR=Zero)  ePWMxLINKCMPB=Not Linked  CMPBUnits=Percentages  CMPBSource=Specify via dialog  CMPBValue_per=50  CMPBValue_clk=32000  enCMPBshadow=Counter equals to zero (CTR=Zero)  ePWMxLINKCMPC=Not Linked  CMPCUnits=Clock cycles  CMPCSource=Specify via dialog  CMPCValue_per=50  CMPCValue_clk=32000  enCMPCshadow=Counter equals to zero (CTR=Zero)  ePWMxLINKCMPD=Not Linked  CMPDUnits=Clock cycles  CMPDSource=Specify via dialog  CMPDValue_per=50  CMPDValue_clk=32000  enCMPDshadow=Counter equals to zero (CTR=Zero)  enableDBePWMxA=on  enableDBePWMxB=on  enhalfcycle=off  DBpolarity=Active high complementary (AHC)  DBedgeDelay=Positive  DBSource_ePWMxA=ePWMxA  DBSource_ePWMxB=ePWMxA  DBPeriodUnits=Clock cycles  DBperiodSource=Specify via dialog  REDperiod=200  FEDperiod=200  REDperiod_sec=0  FEDperiod_sec=0  LoadModeDBRED=Immediate without using shadow  LoadModeDBFED=Immediate without using shadow  adcstartModuleA=on  adcrequestEventA=First event  adcstartEventA=Digital Compare Module A Event 1 start of conversion (DCAEVT1.soc)  adcstartEventA_type2=Counter equals to period (CTR=PRD)  adcstartModuleB=off  adcrequestEventB=First event  adcstartEventB=Counter equals to zero (CTR=Zero)  adcstartEventB_type2=Counter equals to period (CTR=PRD)  intEn=off  intPrd=First event  intSel=Counter equals to zero (CTR=Zero)  intSel_type2=Counter equals to zero (CTR=Zero)  hrpe=off  enHRPWM=off  HRPWM_LoadMode=Counter equals to period (CTR=PRD)  HRPWM_CTLMode=Duty or Period control mode  HRPWM_EDGMode=Both edge  hrpeb=off  enHRPWMB=off  HRPWM_LoadModeB=Counter equals to zero (CTR=ZERO)  HRPWM_CTLModeB=Duty or Period control mode  HRPWM_EDGModeB=Both edge  enHRDBRED=off  enHRDBFED=off  enSFO=on  enautoconv=on  chopperEnable=off  chopperFrequency=1  chopperFirstwidth=1  chopperDuty=12.5%  tripZonesource=Specify via dialog  tzselOSHT1=off  tzselOSHT2=off  tzselOSHT3=off  tzselOSHDCAEV1=off  tzselOSHDCBEV1=off  tzselCBC1=off  tzselCBC2=off  tzselCBC3=off  tzselCBCDCAEV2=off  tzselCBCDCBEV2=off  tzselOSHT4=off  tzselOSHT5=off  tzselOSHT6=off  tzselCBC4=off  tzselCBC5=off  tzselCBC6=off  enTzOstIntr=off  enTzCbcIntr=off  enTzDCAEVT1Intr=off  enTzDCAEVT2Intr=off  enTzDCBEVT1Intr=off  enTzDCBEVT2Intr=off  ePWMxAforced=No action  ePWMxBforced=No action  DCAEVT1forced=No action  DCBEVT1forced=No action  DCAEVT2forced=No action  DCBEVT2forced=No action  dcah=Trip Zone 1 input (TZ1)  dcal=Trip Zone 2 input (TZ2)  dcbh=Trip Zone 1 input (TZ1)  dcbl=Trip Zone 2 input (TZ2)  dcah_type2=GPTRIP1SEL/(TZ1)  dcal_type2=GPTRIP1SEL/(TZ1)  dcbh_type2=GPTRIP1SEL/(TZ1)  dcbl_type2=GPTRIP1SEL/(TZ1)  gendcaevt1=Event disabled  gendcaevt2=Event disabled  gendcbevt1=Event disabled  gendcbevt2=Event disabled  dcaevt1src=DCAEVT1 with sync  dcaevt2src=DCAEVT2 with sync  dcbevt1src=DCBEVT1 with sync  dcbevt2src=DCBEVT2 with sync  pulsesel=Counter equals to zero (CTR=Zero)  blankinv=off  blankoffset=0  blankwidth=0  evsrcsel=Filtered version of DCAEVT1 (DCAEVT1FILT)  encape=off
      settings: LibrarySourceBlock=c2837xDlib/ePWM
  ePWM2 : c2802xlib/ePWM  PwmType=C2000_Type4  useModule=ePWM7  ePWMxLINKTBPRD=Not Linked  periodUnits=Clock cycles  timerSource=Specify via dialog  timerPeriod_clk=4167  timerPeriod_sec=0.0001  tbshadow=Counter equals to zero  countingMode=Up-Down  phaseActiveEnable=Disable  phaseDirection=Count down after sync  phaseActive=0  synchronizationEnable=off  dcaevt1Sync=off  dcbevt1Sync=off  synchronizationOption=Disable  dcbevt1SyncOut=off  dcaevt1SyncOut=off  cmpdSyncOut=off  cmpcSyncOut=off  cmpbSyncOut=off  zeroSyncOut=off  swfSyncOut=off  perSynchronizationOption=Counter equals to period (CTR=PRD)  clockPrescale=1  HSclockPrescale=1  enswap=off  ePWMxAStatus=on  ePWMxAactionLogic1=Set  ePWMxAactionLogic2=Clear  ePWMxAactionLogic3=Clear  ePWMxAactionLogic4=Set  ePWMxAactionLogic5=Do nothing  ePWMxAactionLogic6=Do nothing  ePWMxACSFenable=off  ePWMxACSFvalue=Forcing disable  ePWMxASFreload=Zero  ePWMxBStatus=on  ePWMxBactionLogic1=Set  ePWMxBactionLogic2=Clear  ePWMxBactionLogic3=Do nothing  ePWMxBactionLogic4=Do nothing  ePWMxBactionLogic5=Clear  ePWMxBactionLogic6=Set  ePWMxBCSFenable=off  ePWMxBCSFvalue=Forcing disable  ePWMxBSFreload=Zero  ePWNxBOutWay=off  ePWMxLINKCMPA=Not Linked  CMPAUnits=Percentages  CMPASource=Input port  CMPAValue_per=50  CMPAValue_clk=32000  enCMPAshadow=Counter equals to zero (CTR=Zero)  ePWMxLINKCMPB=Not Linked  CMPBUnits=Percentages  CMPBSource=Input port  CMPBValue_per=50  CMPBValue_clk=32000  enCMPBshadow=Counter equals to zero (CTR=Zero)  ePWMxLINKCMPC=Not Linked  CMPCUnits=Clock cycles  CMPCSource=Specify via dialog  CMPCValue_per=50  CMPCValue_clk=32000  enCMPCshadow=Counter equals to zero (CTR=Zero)  ePWMxLINKCMPD=Not Linked  CMPDUnits=Clock cycles  CMPDSource=Specify via dialog  CMPDValue_per=50  CMPDValue_clk=32000  enCMPDshadow=Counter equals to zero (CTR=Zero)  enableDBePWMxA=off  enableDBePWMxB=off  enhalfcycle=off  DBpolarity=Active high (AH)  DBedgeDelay=Positive  DBSource_ePWMxA=ePWMxA  DBSource_ePWMxB=ePWMxA  DBPeriodUnits=Clock cycles  DBperiodSource=Specify via dialog  REDperiod=0  FEDperiod=0  REDperiod_sec=0  FEDperiod_sec=0  LoadModeDBRED=Immediate without using shadow  LoadModeDBFED=Immediate without using shadow  adcstartModuleA=off  adcrequestEventA=First event  adcstartEventA=Digital Compare Module A Event 1 start of conversion (DCAEVT1.soc)  adcstartEventA_type2=Counter equals to zero (CTR=Zero)  adcstartModuleB=off  adcrequestEventB=First event  adcstartEventB=Counter equals to zero (CTR=Zero)  adcstartEventB_type2=Counter equals to zero (CTR=Zero)  intEn=off  intPrd=First event  intSel=Counter equals to zero (CTR=Zero)  intSel_type2=Counter equals to zero (CTR=Zero)  hrpe=off  enHRPWM=off  HRPWM_LoadMode=Counter equals to period (CTR=PRD)  HRPWM_CTLMode=Duty or Period control mode  HRPWM_EDGMode=Both edge  hrpeb=off  enHRPWMB=off  HRPWM_LoadModeB=Counter equals to zero (CTR=ZERO)  HRPWM_CTLModeB=Duty or Period control mode  HRPWM_EDGModeB=Both edge  enHRDBRED=off  enHRDBFED=off  enSFO=on  enautoconv=on  chopperEnable=off  chopperFrequency=1  chopperFirstwidth=1  chopperDuty=12.5%  tripZonesource=Specify via dialog  tzselOSHT1=off  tzselOSHT2=off  tzselOSHT3=off  tzselOSHDCAEV1=off  tzselOSHDCBEV1=off  tzselCBC1=off  tzselCBC2=off  tzselCBC3=off  tzselCBCDCAEV2=off  tzselCBCDCBEV2=off  tzselOSHT4=off  tzselOSHT5=off  tzselOSHT6=off  tzselCBC4=off  tzselCBC5=off  tzselCBC6=off  enTzOstIntr=off  enTzCbcIntr=off  enTzDCAEVT1Intr=off  enTzDCAEVT2Intr=off  enTzDCBEVT1Intr=off  enTzDCBEVT2Intr=off  ePWMxAforced=No action  ePWMxBforced=No action  DCAEVT1forced=No action  DCBEVT1forced=No action  DCAEVT2forced=No action  DCBEVT2forced=No action  dcah=Trip Zone 1 input (TZ1)  dcal=Trip Zone 2 input (TZ2)  dcbh=Trip Zone 1 input (TZ1)  dcbl=Trip Zone 2 input (TZ2)  dcah_type2=GPTRIP1SEL/(TZ1)  dcal_type2=GPTRIP1SEL/(TZ1)  dcbh_type2=GPTRIP1SEL/(TZ1)  dcbl_type2=GPTRIP1SEL/(TZ1)  gendcaevt1=Event disabled  gendcaevt2=Event disabled  gendcbevt1=Event disabled  gendcbevt2=Event disabled  dcaevt1src=DCAEVT1 with sync  dcaevt2src=DCAEVT2 with sync  dcbevt1src=DCBEVT1 with sync  dcbevt2src=DCBEVT2 with sync  pulsesel=Counter equals to zero (CTR=Zero)  blankinv=off  blankoffset=0  blankwidth=0  evsrcsel=Filtered version of DCAEVT1 (DCAEVT1FILT)  encape=off
      settings: LibrarySourceBlock=c2837xDlib/ePWM
  ePWM20 : c2802xlib/ePWM  PwmType=C2000_Type4  useModule=ePWM5  ePWMxLINKTBPRD=Not Linked  periodUnits=Clock cycles  timerSource=Specify via dialog  timerPeriod_clk=4167  timerPeriod_sec=0.0001  tbshadow=Counter equals to zero  countingMode=Up-Down  phaseActiveEnable=Disable  phaseDirection=Count down after sync  phaseActive=0  synchronizationEnable=off  dcaevt1Sync=off  dcbevt1Sync=off  synchronizationOption=Counter equals to zero (CTR=Zero)  dcbevt1SyncOut=off  dcaevt1SyncOut=off  cmpdSyncOut=off  cmpcSyncOut=off  cmpbSyncOut=off  zeroSyncOut=off  swfSyncOut=off  perSynchronizationOption=Counter equals to period (CTR=PRD)  clockPrescale=1  HSclockPrescale=1  enswap=off  ePWMxAStatus=on  ePWMxAactionLogic1=Set  ePWMxAactionLogic2=Clear  ePWMxAactionLogic3=Clear  ePWMxAactionLogic4=Set  ePWMxAactionLogic5=Do nothing  ePWMxAactionLogic6=Do nothing  ePWMxACSFenable=off  ePWMxACSFvalue=Forcing disable  ePWMxASFreload=Zero  ePWMxBStatus=on  ePWMxBactionLogic1=Set  ePWMxBactionLogic2=Clear  ePWMxBactionLogic3=Do nothing  ePWMxBactionLogic4=Do nothing  ePWMxBactionLogic5=Clear  ePWMxBactionLogic6=Set  ePWMxBCSFenable=off  ePWMxBCSFvalue=Forcing disable  ePWMxBSFreload=Zero  ePWNxBOutWay=off  ePWMxLINKCMPA=Not Linked  CMPAUnits=Percentages  CMPASource=Input port  CMPAValue_per=50  CMPAValue_clk=32000  enCMPAshadow=Counter equals to zero (CTR=Zero)  ePWMxLINKCMPB=Not Linked  CMPBUnits=Percentages  CMPBSource=Specify via dialog  CMPBValue_per=50  CMPBValue_clk=32000  enCMPBshadow=Counter equals to zero (CTR=Zero)  ePWMxLINKCMPC=Not Linked  CMPCUnits=Clock cycles  CMPCSource=Specify via dialog  CMPCValue_per=50  CMPCValue_clk=32000  enCMPCshadow=Counter equals to zero (CTR=Zero)  ePWMxLINKCMPD=Not Linked  CMPDUnits=Clock cycles  CMPDSource=Specify via dialog  CMPDValue_per=50  CMPDValue_clk=32000  enCMPDshadow=Counter equals to zero (CTR=Zero)  enableDBePWMxA=on  enableDBePWMxB=on  enhalfcycle=off  DBpolarity=Active high complementary (AHC)  DBedgeDelay=Positive  DBSource_ePWMxA=ePWMxA  DBSource_ePWMxB=ePWMxA  DBPeriodUnits=Clock cycles  DBperiodSource=Specify via dialog  REDperiod=200  FEDperiod=200  REDperiod_sec=0  FEDperiod_sec=0  LoadModeDBRED=Immediate without using shadow  LoadModeDBFED=Immediate without using shadow  adcstartModuleA=off  adcrequestEventA=First event  adcstartEventA=Digital Compare Module A Event 1 start of conversion (DCAEVT1.soc)  adcstartEventA_type2=Counter equals to zero (CTR=Zero)  adcstartModuleB=off  adcrequestEventB=First event  adcstartEventB=Counter equals to zero (CTR=Zero)  adcstartEventB_type2=Counter equals to zero (CTR=Zero)  intEn=off  intPrd=First event  intSel=Counter equals to zero (CTR=Zero)  intSel_type2=Counter equals to zero (CTR=Zero)  hrpe=off  enHRPWM=off  HRPWM_LoadMode=Counter equals to period (CTR=PRD)  HRPWM_CTLMode=Duty or Period control mode  HRPWM_EDGMode=Both edge  hrpeb=off  enHRPWMB=off  HRPWM_LoadModeB=Counter equals to zero (CTR=ZERO)  HRPWM_CTLModeB=Duty or Period control mode  HRPWM_EDGModeB=Both edge  enHRDBRED=off  enHRDBFED=off  enSFO=on  enautoconv=on  chopperEnable=off  chopperFrequency=1  chopperFirstwidth=1  chopperDuty=12.5%  tripZonesource=Specify via dialog  tzselOSHT1=off  tzselOSHT2=off  tzselOSHT3=off  tzselOSHDCAEV1=off  tzselOSHDCBEV1=off  tzselCBC1=off  tzselCBC2=off  tzselCBC3=off  tzselCBCDCAEV2=off  tzselCBCDCBEV2=off  tzselOSHT4=off  tzselOSHT5=off  tzselOSHT6=off  tzselCBC4=off  tzselCBC5=off  tzselCBC6=off  enTzOstIntr=off  enTzCbcIntr=off  enTzDCAEVT1Intr=off  enTzDCAEVT2Intr=off  enTzDCBEVT1Intr=off  enTzDCBEVT2Intr=off  ePWMxAforced=No action  ePWMxBforced=No action  DCAEVT1forced=No action  DCBEVT1forced=No action  DCAEVT2forced=No action  DCBEVT2forced=No action  dcah=Trip Zone 1 input (TZ1)  dcal=Trip Zone 2 input (TZ2)  dcbh=Trip Zone 1 input (TZ1)  dcbl=Trip Zone 2 input (TZ2)  dcah_type2=GPTRIP1SEL/(TZ1)  dcal_type2=GPTRIP1SEL/(TZ1)  dcbh_type2=GPTRIP1SEL/(TZ1)  dcbl_type2=GPTRIP1SEL/(TZ1)  gendcaevt1=Event disabled  gendcaevt2=Event disabled  gendcbevt1=Event disabled  gendcbevt2=Event disabled  dcaevt1src=DCAEVT1 with sync  dcaevt2src=DCAEVT2 with sync  dcbevt1src=DCBEVT1 with sync  dcbevt2src=DCBEVT2 with sync  pulsesel=Counter equals to zero (CTR=Zero)  blankinv=off  blankoffset=0  blankwidth=0  evsrcsel=Filtered version of DCAEVT1 (DCAEVT1FILT)  encape=off
      settings: LibrarySourceBlock=c2837xDlib/ePWM
  ePWM21 : c2802xlib/ePWM  PwmType=C2000_Type4  useModule=ePWM2  ePWMxLINKTBPRD=Not Linked  periodUnits=Clock cycles  timerSource=Specify via dialog  timerPeriod_clk=4167  timerPeriod_sec=0.0001  tbshadow=Counter equals to zero  countingMode=Up-Down  phaseActiveEnable=Disable  phaseDirection=Count down after sync  phaseActive=0  synchronizationEnable=off  dcaevt1Sync=off  dcbevt1Sync=off  synchronizationOption=Counter equals to zero (CTR=Zero)  dcbevt1SyncOut=off  dcaevt1SyncOut=off  cmpdSyncOut=off  cmpcSyncOut=off  cmpbSyncOut=off  zeroSyncOut=off  swfSyncOut=off  perSynchronizationOption=Counter equals to period (CTR=PRD)  clockPrescale=1  HSclockPrescale=1  enswap=off  ePWMxAStatus=on  ePWMxAactionLogic1=Set  ePWMxAactionLogic2=Clear  ePWMxAactionLogic3=Clear  ePWMxAactionLogic4=Set  ePWMxAactionLogic5=Do nothing  ePWMxAactionLogic6=Do nothing  ePWMxACSFenable=off  ePWMxACSFvalue=Forcing disable  ePWMxASFreload=Zero  ePWMxBStatus=on  ePWMxBactionLogic1=Set  ePWMxBactionLogic2=Clear  ePWMxBactionLogic3=Do nothing  ePWMxBactionLogic4=Do nothing  ePWMxBactionLogic5=Clear  ePWMxBactionLogic6=Set  ePWMxBCSFenable=off  ePWMxBCSFvalue=Forcing disable  ePWMxBSFreload=Zero  ePWNxBOutWay=off  ePWMxLINKCMPA=Not Linked  CMPAUnits=Percentages  CMPASource=Input port  CMPAValue_per=50  CMPAValue_clk=32000  enCMPAshadow=Counter equals to zero (CTR=Zero)  ePWMxLINKCMPB=Not Linked  CMPBUnits=Percentages  CMPBSource=Input port  CMPBValue_per=50  CMPBValue_clk=32000  enCMPBshadow=Counter equals to zero (CTR=Zero)  ePWMxLINKCMPC=Not Linked  CMPCUnits=Clock cycles  CMPCSource=Specify via dialog  CMPCValue_per=50  CMPCValue_clk=32000  enCMPCshadow=Counter equals to zero (CTR=Zero)  ePWMxLINKCMPD=Not Linked  CMPDUnits=Clock cycles  CMPDSource=Specify via dialog  CMPDValue_per=50  CMPDValue_clk=32000  enCMPDshadow=Counter equals to zero (CTR=Zero)  enableDBePWMxA=off  enableDBePWMxB=off  enhalfcycle=off  DBpolarity=Active high complementary (AHC)  DBedgeDelay=Positive  DBSource_ePWMxA=ePWMxA  DBSource_ePWMxB=ePWMxA  DBPeriodUnits=Clock cycles  DBperiodSource=Specify via dialog  REDperiod=200  FEDperiod=200  REDperiod_sec=0  FEDperiod_sec=0  LoadModeDBRED=Immediate without using shadow  LoadModeDBFED=Immediate without using shadow  adcstartModuleA=off  adcrequestEventA=First event  adcstartEventA=Digital Compare Module A Event 1 start of conversion (DCAEVT1.soc)  adcstartEventA_type2=Counter equals to zero (CTR=Zero)  adcstartModuleB=off  adcrequestEventB=First event  adcstartEventB=Counter equals to zero (CTR=Zero)  adcstartEventB_type2=Counter equals to zero (CTR=Zero)  intEn=off  intPrd=First event  intSel=Counter equals to zero (CTR=Zero)  intSel_type2=Counter equals to zero (CTR=Zero)  hrpe=off  enHRPWM=off  HRPWM_LoadMode=Counter equals to period (CTR=PRD)  HRPWM_CTLMode=Duty or Period control mode  HRPWM_EDGMode=Both edge  hrpeb=off  enHRPWMB=off  HRPWM_LoadModeB=Counter equals to zero (CTR=ZERO)  HRPWM_CTLModeB=Duty or Period control mode  HRPWM_EDGModeB=Both edge  enHRDBRED=off  enHRDBFED=off  enSFO=on  enautoconv=on  chopperEnable=off  chopperFrequency=1  chopperFirstwidth=1  chopperDuty=12.5%  tripZonesource=Specify via dialog  tzselOSHT1=off  tzselOSHT2=off  tzselOSHT3=off  tzselOSHDCAEV1=off  tzselOSHDCBEV1=off  tzselCBC1=off  tzselCBC2=off  tzselCBC3=off  tzselCBCDCAEV2=off  tzselCBCDCBEV2=off  tzselOSHT4=off  tzselOSHT5=off  tzselOSHT6=off  tzselCBC4=off  tzselCBC5=off  tzselCBC6=off  enTzOstIntr=off  enTzCbcIntr=off  enTzDCAEVT1Intr=off  enTzDCAEVT2Intr=off  enTzDCBEVT1Intr=off  enTzDCBEVT2Intr=off  ePWMxAforced=No action  ePWMxBforced=No action  DCAEVT1forced=No action  DCBEVT1forced=No action  DCAEVT2forced=No action  DCBEVT2forced=No action  dcah=Trip Zone 1 input (TZ1)  dcal=Trip Zone 2 input (TZ2)  dcbh=Trip Zone 1 input (TZ1)  dcbl=Trip Zone 2 input (TZ2)  dcah_type2=GPTRIP1SEL/(TZ1)  dcal_type2=GPTRIP1SEL/(TZ1)  dcbh_type2=GPTRIP1SEL/(TZ1)  dcbl_type2=GPTRIP1SEL/(TZ1)  gendcaevt1=Event disabled  gendcaevt2=Event disabled  gendcbevt1=Event disabled  gendcbevt2=Event disabled  dcaevt1src=DCAEVT1 with sync  dcaevt2src=DCAEVT2 with sync  dcbevt1src=DCBEVT1 with sync  dcbevt2src=DCBEVT2 with sync  pulsesel=Counter equals to zero (CTR=Zero)  blankinv=off  blankoffset=0  blankwidth=0  evsrcsel=Filtered version of DCAEVT1 (DCAEVT1FILT)  encape=off
      settings: LibrarySourceBlock=c2837xDlib/ePWM
  ePWM22 : c2802xlib/ePWM  PwmType=C2000_Type4  useModule=ePWM3  ePWMxLINKTBPRD=Not Linked  periodUnits=Clock cycles  timerSource=Specify via dialog  timerPeriod_clk=4167  timerPeriod_sec=0.0001  tbshadow=Counter equals to zero  countingMode=Up-Down  phaseActiveEnable=Disable  phaseDirection=Count down after sync  phaseActive=0  synchronizationEnable=off  dcaevt1Sync=off  dcbevt1Sync=off  synchronizationOption=Counter equals to zero (CTR=Zero)  dcbevt1SyncOut=off  dcaevt1SyncOut=off  cmpdSyncOut=off  cmpcSyncOut=off  cmpbSyncOut=off  zeroSyncOut=off  swfSyncOut=off  perSynchronizationOption=Counter equals to period (CTR=PRD)  clockPrescale=1  HSclockPrescale=1  enswap=off  ePWMxAStatus=on  ePWMxAactionLogic1=Set  ePWMxAactionLogic2=Clear  ePWMxAactionLogic3=Clear  ePWMxAactionLogic4=Set  ePWMxAactionLogic5=Do nothing  ePWMxAactionLogic6=Do nothing  ePWMxACSFenable=off  ePWMxACSFvalue=Forcing disable  ePWMxASFreload=Zero  ePWMxBStatus=on  ePWMxBactionLogic1=Set  ePWMxBactionLogic2=Clear  ePWMxBactionLogic3=Do nothing  ePWMxBactionLogic4=Do nothing  ePWMxBactionLogic5=Clear  ePWMxBactionLogic6=Set  ePWMxBCSFenable=off  ePWMxBCSFvalue=Forcing disable  ePWMxBSFreload=Zero  ePWNxBOutWay=off  ePWMxLINKCMPA=Not Linked  CMPAUnits=Percentages  CMPASource=Input port  CMPAValue_per=50  CMPAValue_clk=32000  enCMPAshadow=Counter equals to zero (CTR=Zero)  ePWMxLINKCMPB=Not Linked  CMPBUnits=Percentages  CMPBSource=Specify via dialog  CMPBValue_per=50  CMPBValue_clk=32000  enCMPBshadow=Counter equals to zero (CTR=Zero)  ePWMxLINKCMPC=Not Linked  CMPCUnits=Clock cycles  CMPCSource=Specify via dialog  CMPCValue_per=50  CMPCValue_clk=32000  enCMPCshadow=Counter equals to zero (CTR=Zero)  ePWMxLINKCMPD=Not Linked  CMPDUnits=Clock cycles  CMPDSource=Specify via dialog  CMPDValue_per=50  CMPDValue_clk=32000  enCMPDshadow=Counter equals to zero (CTR=Zero)  enableDBePWMxA=on  enableDBePWMxB=on  enhalfcycle=off  DBpolarity=Active high complementary (AHC)  DBedgeDelay=Positive  DBSource_ePWMxA=ePWMxA  DBSource_ePWMxB=ePWMxA  DBPeriodUnits=Clock cycles  DBperiodSource=Specify via dialog  REDperiod=200  FEDperiod=200  REDperiod_sec=0  FEDperiod_sec=0  LoadModeDBRED=Immediate without using shadow  LoadModeDBFED=Immediate without using shadow  adcstartModuleA=off  adcrequestEventA=First event  adcstartEventA=Digital Compare Module A Event 1 start of conversion (DCAEVT1.soc)  adcstartEventA_type2=Counter equals to zero (CTR=Zero)  adcstartModuleB=off  adcrequestEventB=First event  adcstartEventB=Counter equals to zero (CTR=Zero)  adcstartEventB_type2=Counter equals to zero (CTR=Zero)  intEn=off  intPrd=First event  intSel=Counter equals to zero (CTR=Zero)  intSel_type2=Counter equals to zero (CTR=Zero)  hrpe=off  enHRPWM=off  HRPWM_LoadMode=Counter equals to period (CTR=PRD)  HRPWM_CTLMode=Duty or Period control mode  HRPWM_EDGMode=Both edge  hrpeb=off  enHRPWMB=off  HRPWM_LoadModeB=Counter equals to zero (CTR=ZERO)  HRPWM_CTLModeB=Duty or Period control mode  HRPWM_EDGModeB=Both edge  enHRDBRED=off  enHRDBFED=off  enSFO=on  enautoconv=on  chopperEnable=off  chopperFrequency=1  chopperFirstwidth=1  chopperDuty=12.5%  tripZonesource=Specify via dialog  tzselOSHT1=off  tzselOSHT2=off  tzselOSHT3=off  tzselOSHDCAEV1=off  tzselOSHDCBEV1=off  tzselCBC1=off  tzselCBC2=off  tzselCBC3=off  tzselCBCDCAEV2=off  tzselCBCDCBEV2=off  tzselOSHT4=off  tzselOSHT5=off  tzselOSHT6=off  tzselCBC4=off  tzselCBC5=off  tzselCBC6=off  enTzOstIntr=off  enTzCbcIntr=off  enTzDCAEVT1Intr=off  enTzDCAEVT2Intr=off  enTzDCBEVT1Intr=off  enTzDCBEVT2Intr=off  ePWMxAforced=No action  ePWMxBforced=No action  DCAEVT1forced=No action  DCBEVT1forced=No action  DCAEVT2forced=No action  DCBEVT2forced=No action  dcah=Trip Zone 1 input (TZ1)  dcal=Trip Zone 2 input (TZ2)  dcbh=Trip Zone 1 input (TZ1)  dcbl=Trip Zone 2 input (TZ2)  dcah_type2=GPTRIP1SEL/(TZ1)  dcal_type2=GPTRIP1SEL/(TZ1)  dcbh_type2=GPTRIP1SEL/(TZ1)  dcbl_type2=GPTRIP1SEL/(TZ1)  gendcaevt1=Event disabled  gendcaevt2=Event disabled  gendcbevt1=Event disabled  gendcbevt2=Event disabled  dcaevt1src=DCAEVT1 with sync  dcaevt2src=DCAEVT2 with sync  dcbevt1src=DCBEVT1 with sync  dcbevt2src=DCBEVT2 with sync  pulsesel=Counter equals to zero (CTR=Zero)  blankinv=off  blankoffset=0  blankwidth=0  evsrcsel=Filtered version of DCAEVT1 (DCAEVT1FILT)  encape=off
      settings: LibrarySourceBlock=c2837xDlib/ePWM
  ePWM3 : c2802xlib/ePWM  Commented=on  PwmType=C2000_Type4  useModule=ePWM2  ePWMxLINKTBPRD=Not Linked  periodUnits=Clock cycles  timerSource=Specify via dialog  timerPeriod_clk=4166  timerPeriod_sec=0.0001  tbshadow=Counter equals to zero  countingMode=Up-Down  phaseActiveEnable=Disable  phaseDirection=Count down after sync  phaseActive=0  synchronizationEnable=off  dcaevt1Sync=off  dcbevt1Sync=off  synchronizationOption=Disable  dcbevt1SyncOut=off  dcaevt1SyncOut=off  cmpdSyncOut=off  cmpcSyncOut=off  cmpbSyncOut=off  zeroSyncOut=off  swfSyncOut=off  perSynchronizationOption=Counter equals to period (CTR=PRD)  clockPrescale=1  HSclockPrescale=1  enswap=off  ePWMxAStatus=on  ePWMxAactionLogic1=Set  ePWMxAactionLogic2=Clear  ePWMxAactionLogic3=Clear  ePWMxAactionLogic4=Set  ePWMxAactionLogic5=Do nothing  ePWMxAactionLogic6=Do nothing  ePWMxACSFenable=off  ePWMxACSFvalue=Forcing disable  ePWMxASFreload=Zero  ePWMxBStatus=on  ePWMxBactionLogic1=Set  ePWMxBactionLogic2=Clear  ePWMxBactionLogic3=Do nothing  ePWMxBactionLogic4=Do nothing  ePWMxBactionLogic5=Clear  ePWMxBactionLogic6=Set  ePWMxBCSFenable=off  ePWMxBCSFvalue=Forcing disable  ePWMxBSFreload=Zero  ePWNxBOutWay=off  ePWMxLINKCMPA=Not Linked  CMPAUnits=Percentages  CMPASource=Input port  CMPAValue_per=50  CMPAValue_clk=32000  enCMPAshadow=Counter equals to zero (CTR=Zero)  ePWMxLINKCMPB=Not Linked  CMPBUnits=Percentages  CMPBSource=Input port  CMPBValue_per=50  CMPBValue_clk=32000  enCMPBshadow=Counter equals to zero (CTR=Zero)  ePWMxLINKCMPC=Not Linked  CMPCUnits=Clock cycles  CMPCSource=Specify via dialog  CMPCValue_per=50  CMPCValue_clk=32000  enCMPCshadow=Counter equals to zero (CTR=Zero)  ePWMxLINKCMPD=Not Linked  CMPDUnits=Clock cycles  CMPDSource=Specify via dialog  CMPDValue_per=50  CMPDValue_clk=32000  enCMPDshadow=Counter equals to zero (CTR=Zero)  enableDBePWMxA=off  enableDBePWMxB=off  enhalfcycle=off  DBpolarity=Active high (AH)  DBedgeDelay=Positive  DBSource_ePWMxA=ePWMxA  DBSource_ePWMxB=ePWMxA  DBPeriodUnits=Clock cycles  DBperiodSource=Specify via dialog  REDperiod=0  FEDperiod=0  REDperiod_sec=0  FEDperiod_sec=0  LoadModeDBRED=Immediate without using shadow  LoadModeDBFED=Immediate without using shadow  adcstartModuleA=off  adcrequestEventA=First event  adcstartEventA=Digital Compare Module A Event 1 start of conversion (DCAEVT1.soc)  adcstartEventA_type2=Counter equals to zero (CTR=Zero)  adcstartModuleB=off  adcrequestEventB=First event  adcstartEventB=Counter equals to zero (CTR=Zero)  adcstartEventB_type2=Counter equals to zero (CTR=Zero)  intEn=off  intPrd=First event  intSel=Counter equals to zero (CTR=Zero)  intSel_type2=Counter equals to zero (CTR=Zero)  hrpe=off  enHRPWM=off  HRPWM_LoadMode=Counter equals to period (CTR=PRD)  HRPWM_CTLMode=Duty or Period control mode  HRPWM_EDGMode=Both edge  hrpeb=off  enHRPWMB=off  HRPWM_LoadModeB=Counter equals to zero (CTR=ZERO)  HRPWM_CTLModeB=Duty or Period control mode  HRPWM_EDGModeB=Both edge  enHRDBRED=off  enHRDBFED=off  enSFO=on  enautoconv=on  chopperEnable=off  chopperFrequency=1  chopperFirstwidth=1  chopperDuty=12.5%  tripZonesource=Specify via dialog  tzselOSHT1=off  tzselOSHT2=off  tzselOSHT3=off  tzselOSHDCAEV1=off  tzselOSHDCBEV1=off  tzselCBC1=off  tzselCBC2=off  tzselCBC3=off  tzselCBCDCAEV2=off  tzselCBCDCBEV2=off  tzselOSHT4=off  tzselOSHT5=off  tzselOSHT6=off  tzselCBC4=off  tzselCBC5=off  tzselCBC6=off  enTzOstIntr=off  enTzCbcIntr=off  enTzDCAEVT1Intr=off  enTzDCAEVT2Intr=off  enTzDCBEVT1Intr=off  enTzDCBEVT2Intr=off  ePWMxAforced=No action  ePWMxBforced=No action  DCAEVT1forced=No action  DCBEVT1forced=No action  DCAEVT2forced=No action  DCBEVT2forced=No action  dcah=Trip Zone 1 input (TZ1)  dcal=Trip Zone 2 input (TZ2)  dcbh=Trip Zone 1 input (TZ1)  dcbl=Trip Zone 2 input (TZ2)  dcah_type2=GPTRIP1SEL/(TZ1)  dcal_type2=GPTRIP1SEL/(TZ1)  dcbh_type2=GPTRIP1SEL/(TZ1)  dcbl_type2=GPTRIP1SEL/(TZ1)  gendcaevt1=Event disabled  gendcaevt2=Event disabled  gendcbevt1=Event disabled  gendcbevt2=Event disabled  dcaevt1src=DCAEVT1 with sync  dcaevt2src=DCAEVT2 with sync  dcbevt1src=DCBEVT1 with sync  dcbevt2src=DCBEVT2 with sync  pulsesel=Counter equals to zero (CTR=Zero)  blankinv=off  blankoffset=0  blankwidth=0  evsrcsel=Filtered version of DCAEVT1 (DCAEVT1FILT)  encape=off
      settings: LibrarySourceBlock=c2837xDlib/ePWM
  ePWM4 : c2802xlib/ePWM  Commented=on  PwmType=C2000_Type4  useModule=ePWM3  ePWMxLINKTBPRD=Not Linked  periodUnits=Clock cycles  timerSource=Specify via dialog  timerPeriod_clk=4166  timerPeriod_sec=0.0001  tbshadow=Counter equals to zero  countingMode=Up-Down  phaseActiveEnable=Disable  phaseDirection=Count down after sync  phaseActive=0  synchronizationEnable=off  dcaevt1Sync=off  dcbevt1Sync=off  synchronizationOption=Disable  dcbevt1SyncOut=off  dcaevt1SyncOut=off  cmpdSyncOut=off  cmpcSyncOut=off  cmpbSyncOut=off  zeroSyncOut=off  swfSyncOut=off  perSynchronizationOption=Counter equals to period (CTR=PRD)  clockPrescale=1  HSclockPrescale=1  enswap=off  ePWMxAStatus=on  ePWMxAactionLogic1=Set  ePWMxAactionLogic2=Clear  ePWMxAactionLogic3=Clear  ePWMxAactionLogic4=Set  ePWMxAactionLogic5=Do nothing  ePWMxAactionLogic6=Do nothing  ePWMxACSFenable=off  ePWMxACSFvalue=Forcing disable  ePWMxASFreload=Zero  ePWMxBStatus=on  ePWMxBactionLogic1=Set  ePWMxBactionLogic2=Clear  ePWMxBactionLogic3=Do nothing  ePWMxBactionLogic4=Do nothing  ePWMxBactionLogic5=Clear  ePWMxBactionLogic6=Set  ePWMxBCSFenable=off  ePWMxBCSFvalue=Forcing disable  ePWMxBSFreload=Zero  ePWNxBOutWay=off  ePWMxLINKCMPA=Not Linked  CMPAUnits=Percentages  CMPASource=Input port  CMPAValue_per=50  CMPAValue_clk=32000  enCMPAshadow=Counter equals to zero (CTR=Zero)  ePWMxLINKCMPB=Not Linked  CMPBUnits=Percentages  CMPBSource=Input port  CMPBValue_per=50  CMPBValue_clk=32000  enCMPBshadow=Counter equals to zero (CTR=Zero)  ePWMxLINKCMPC=Not Linked  CMPCUnits=Clock cycles  CMPCSource=Specify via dialog  CMPCValue_per=50  CMPCValue_clk=32000  enCMPCshadow=Counter equals to zero (CTR=Zero)  ePWMxLINKCMPD=Not Linked  CMPDUnits=Clock cycles  CMPDSource=Specify via dialog  CMPDValue_per=50  CMPDValue_clk=32000  enCMPDshadow=Counter equals to zero (CTR=Zero)  enableDBePWMxA=off  enableDBePWMxB=off  enhalfcycle=off  DBpolarity=Active high (AH)  DBedgeDelay=Positive  DBSource_ePWMxA=ePWMxA  DBSource_ePWMxB=ePWMxA  DBPeriodUnits=Clock cycles  DBperiodSource=Specify via dialog  REDperiod=0  FEDperiod=0  REDperiod_sec=0  FEDperiod_sec=0  LoadModeDBRED=Immediate without using shadow  LoadModeDBFED=Immediate without using shadow  adcstartModuleA=off  adcrequestEventA=First event  adcstartEventA=Digital Compare Module A Event 1 start of conversion (DCAEVT1.soc)  adcstartEventA_type2=Counter equals to zero (CTR=Zero)  adcstartModuleB=off  adcrequestEventB=First event  adcstartEventB=Counter equals to zero (CTR=Zero)  adcstartEventB_type2=Counter equals to zero (CTR=Zero)  intEn=off  intPrd=First event  intSel=Counter equals to zero (CTR=Zero)  intSel_type2=Counter equals to zero (CTR=Zero)  hrpe=off  enHRPWM=off  HRPWM_LoadMode=Counter equals to period (CTR=PRD)  HRPWM_CTLMode=Duty or Period control mode  HRPWM_EDGMode=Both edge  hrpeb=off  enHRPWMB=off  HRPWM_LoadModeB=Counter equals to zero (CTR=ZERO)  HRPWM_CTLModeB=Duty or Period control mode  HRPWM_EDGModeB=Both edge  enHRDBRED=off  enHRDBFED=off  enSFO=on  enautoconv=on  chopperEnable=off  chopperFrequency=1  chopperFirstwidth=1  chopperDuty=12.5%  tripZonesource=Specify via dialog  tzselOSHT1=off  tzselOSHT2=off  tzselOSHT3=off  tzselOSHDCAEV1=off  tzselOSHDCBEV1=off  tzselCBC1=off  tzselCBC2=off  tzselCBC3=off  tzselCBCDCAEV2=off  tzselCBCDCBEV2=off  tzselOSHT4=off  tzselOSHT5=off  tzselOSHT6=off  tzselCBC4=off  tzselCBC5=off  tzselCBC6=off  enTzOstIntr=off  enTzCbcIntr=off  enTzDCAEVT1Intr=off  enTzDCAEVT2Intr=off  enTzDCBEVT1Intr=off  enTzDCBEVT2Intr=off  ePWMxAforced=No action  ePWMxBforced=No action  DCAEVT1forced=No action  DCBEVT1forced=No action  DCAEVT2forced=No action  DCBEVT2forced=No action  dcah=Trip Zone 1 input (TZ1)  dcal=Trip Zone 2 input (TZ2)  dcbh=Trip Zone 1 input (TZ1)  dcbl=Trip Zone 2 input (TZ2)  dcah_type2=GPTRIP1SEL/(TZ1)  dcal_type2=GPTRIP1SEL/(TZ1)  dcbh_type2=GPTRIP1SEL/(TZ1)  dcbl_type2=GPTRIP1SEL/(TZ1)  gendcaevt1=Event disabled  gendcaevt2=Event disabled  gendcbevt1=Event disabled  gendcbevt2=Event disabled  dcaevt1src=DCAEVT1 with sync  dcaevt2src=DCAEVT2 with sync  dcbevt1src=DCBEVT1 with sync  dcbevt2src=DCBEVT2 with sync  pulsesel=Counter equals to zero (CTR=Zero)  blankinv=off  blankoffset=0  blankwidth=0  evsrcsel=Filtered version of DCAEVT1 (DCAEVT1FILT)  encape=off
      settings: LibrarySourceBlock=c2837xDlib/ePWM
  ePWM5 : c2802xlib/ePWM  Commented=on  PwmType=C2000_Type4  useModule=ePWM4  ePWMxLINKTBPRD=Not Linked  periodUnits=Clock cycles  timerSource=Specify via dialog  timerPeriod_clk=4166  timerPeriod_sec=0.0001  tbshadow=Counter equals to zero  countingMode=Up-Down  phaseActiveEnable=Disable  phaseDirection=Count down after sync  phaseActive=0  synchronizationEnable=off  dcaevt1Sync=off  dcbevt1Sync=off  synchronizationOption=Disable  dcbevt1SyncOut=off  dcaevt1SyncOut=off  cmpdSyncOut=off  cmpcSyncOut=off  cmpbSyncOut=off  zeroSyncOut=off  swfSyncOut=off  perSynchronizationOption=Counter equals to period (CTR=PRD)  clockPrescale=1  HSclockPrescale=1  enswap=off  ePWMxAStatus=on  ePWMxAactionLogic1=Set  ePWMxAactionLogic2=Clear  ePWMxAactionLogic3=Clear  ePWMxAactionLogic4=Set  ePWMxAactionLogic5=Do nothing  ePWMxAactionLogic6=Do nothing  ePWMxACSFenable=off  ePWMxACSFvalue=Forcing disable  ePWMxASFreload=Zero  ePWMxBStatus=on  ePWMxBactionLogic1=Set  ePWMxBactionLogic2=Clear  ePWMxBactionLogic3=Do nothing  ePWMxBactionLogic4=Do nothing  ePWMxBactionLogic5=Clear  ePWMxBactionLogic6=Set  ePWMxBCSFenable=off  ePWMxBCSFvalue=Forcing disable  ePWMxBSFreload=Zero  ePWNxBOutWay=off  ePWMxLINKCMPA=Not Linked  CMPAUnits=Percentages  CMPASource=Input port  CMPAValue_per=50  CMPAValue_clk=32000  enCMPAshadow=Counter equals to zero (CTR=Zero)  ePWMxLINKCMPB=Not Linked  CMPBUnits=Percentages  CMPBSource=Input port  CMPBValue_per=50  CMPBValue_clk=32000  enCMPBshadow=Counter equals to zero (CTR=Zero)  ePWMxLINKCMPC=Not Linked  CMPCUnits=Clock cycles  CMPCSource=Specify via dialog  CMPCValue_per=50  CMPCValue_clk=32000  enCMPCshadow=Counter equals to zero (CTR=Zero)  ePWMxLINKCMPD=Not Linked  CMPDUnits=Clock cycles  CMPDSource=Specify via dialog  CMPDValue_per=50  CMPDValue_clk=32000  enCMPDshadow=Counter equals to zero (CTR=Zero)  enableDBePWMxA=off  enableDBePWMxB=off  enhalfcycle=off  DBpolarity=Active high (AH)  DBedgeDelay=Positive  DBSource_ePWMxA=ePWMxA  DBSource_ePWMxB=ePWMxA  DBPeriodUnits=Clock cycles  DBperiodSource=Specify via dialog  REDperiod=0  FEDperiod=0  REDperiod_sec=0  FEDperiod_sec=0  LoadModeDBRED=Immediate without using shadow  LoadModeDBFED=Immediate without using shadow  adcstartModuleA=off  adcrequestEventA=First event  adcstartEventA=Digital Compare Module A Event 1 start of conversion (DCAEVT1.soc)  adcstartEventA_type2=Counter equals to zero (CTR=Zero)  adcstartModuleB=off  adcrequestEventB=First event  adcstartEventB=Counter equals to zero (CTR=Zero)  adcstartEventB_type2=Counter equals to zero (CTR=Zero)  intEn=off  intPrd=First event  intSel=Counter equals to zero (CTR=Zero)  intSel_type2=Counter equals to zero (CTR=Zero)  hrpe=off  enHRPWM=off  HRPWM_LoadMode=Counter equals to period (CTR=PRD)  HRPWM_CTLMode=Duty or Period control mode  HRPWM_EDGMode=Both edge  hrpeb=off  enHRPWMB=off  HRPWM_LoadModeB=Counter equals to zero (CTR=ZERO)  HRPWM_CTLModeB=Duty or Period control mode  HRPWM_EDGModeB=Both edge  enHRDBRED=off  enHRDBFED=off  enSFO=on  enautoconv=on  chopperEnable=off  chopperFrequency=1  chopperFirstwidth=1  chopperDuty=12.5%  tripZonesource=Specify via dialog  tzselOSHT1=off  tzselOSHT2=off  tzselOSHT3=off  tzselOSHDCAEV1=off  tzselOSHDCBEV1=off  tzselCBC1=off  tzselCBC2=off  tzselCBC3=off  tzselCBCDCAEV2=off  tzselCBCDCBEV2=off  tzselOSHT4=off  tzselOSHT5=off  tzselOSHT6=off  tzselCBC4=off  tzselCBC5=off  tzselCBC6=off  enTzOstIntr=off  enTzCbcIntr=off  enTzDCAEVT1Intr=off  enTzDCAEVT2Intr=off  enTzDCBEVT1Intr=off  enTzDCBEVT2Intr=off  ePWMxAforced=No action  ePWMxBforced=No action  DCAEVT1forced=No action  DCBEVT1forced=No action  DCAEVT2forced=No action  DCBEVT2forced=No action  dcah=Trip Zone 1 input (TZ1)  dcal=Trip Zone 2 input (TZ2)  dcbh=Trip Zone 1 input (TZ1)  dcbl=Trip Zone 2 input (TZ2)  dcah_type2=GPTRIP1SEL/(TZ1)  dcal_type2=GPTRIP1SEL/(TZ1)  dcbh_type2=GPTRIP1SEL/(TZ1)  dcbl_type2=GPTRIP1SEL/(TZ1)  gendcaevt1=Event disabled  gendcaevt2=Event disabled  gendcbevt1=Event disabled  gendcbevt2=Event disabled  dcaevt1src=DCAEVT1 with sync  dcaevt2src=DCAEVT2 with sync  dcbevt1src=DCBEVT1 with sync  dcbevt2src=DCBEVT2 with sync  pulsesel=Counter equals to zero (CTR=Zero)  blankinv=off  blankoffset=0  blankwidth=0  evsrcsel=Filtered version of DCAEVT1 (DCAEVT1FILT)  encape=off
      settings: LibrarySourceBlock=c2837xDlib/ePWM
  ePWM6 : c2802xlib/ePWM  Commented=on  PwmType=C2000_Type4  useModule=ePWM5  ePWMxLINKTBPRD=Not Linked  periodUnits=Clock cycles  timerSource=Specify via dialog  timerPeriod_clk=4166  timerPeriod_sec=0.0001  tbshadow=Counter equals to zero  countingMode=Up-Down  phaseActiveEnable=Disable  phaseDirection=Count down after sync  phaseActive=0  synchronizationEnable=off  dcaevt1Sync=off  dcbevt1Sync=off  synchronizationOption=Disable  dcbevt1SyncOut=off  dcaevt1SyncOut=off  cmpdSyncOut=off  cmpcSyncOut=off  cmpbSyncOut=off  zeroSyncOut=off  swfSyncOut=off  perSynchronizationOption=Counter equals to period (CTR=PRD)  clockPrescale=1  HSclockPrescale=1  enswap=off  ePWMxAStatus=on  ePWMxAactionLogic1=Set  ePWMxAactionLogic2=Clear  ePWMxAactionLogic3=Clear  ePWMxAactionLogic4=Set  ePWMxAactionLogic5=Do nothing  ePWMxAactionLogic6=Do nothing  ePWMxACSFenable=off  ePWMxACSFvalue=Forcing disable  ePWMxASFreload=Zero  ePWMxBStatus=on  ePWMxBactionLogic1=Set  ePWMxBactionLogic2=Clear  ePWMxBactionLogic3=Do nothing  ePWMxBactionLogic4=Do nothing  ePWMxBactionLogic5=Clear  ePWMxBactionLogic6=Set  ePWMxBCSFenable=off  ePWMxBCSFvalue=Forcing disable  ePWMxBSFreload=Zero  ePWNxBOutWay=off  ePWMxLINKCMPA=Not Linked  CMPAUnits=Percentages  CMPASource=Input port  CMPAValue_per=50  CMPAValue_clk=32000  enCMPAshadow=Counter equals to zero (CTR=Zero)  ePWMxLINKCMPB=Not Linked  CMPBUnits=Percentages  CMPBSource=Input port  CMPBValue_per=50  CMPBValue_clk=32000  enCMPBshadow=Counter equals to zero (CTR=Zero)  ePWMxLINKCMPC=Not Linked  CMPCUnits=Clock cycles  CMPCSource=Specify via dialog  CMPCValue_per=50  CMPCValue_clk=32000  enCMPCshadow=Counter equals to zero (CTR=Zero)  ePWMxLINKCMPD=Not Linked  CMPDUnits=Clock cycles  CMPDSource=Specify via dialog  CMPDValue_per=50  CMPDValue_clk=32000  enCMPDshadow=Counter equals to zero (CTR=Zero)  enableDBePWMxA=off  enableDBePWMxB=off  enhalfcycle=off  DBpolarity=Active high (AH)  DBedgeDelay=Positive  DBSource_ePWMxA=ePWMxA  DBSource_ePWMxB=ePWMxA  DBPeriodUnits=Clock cycles  DBperiodSource=Specify via dialog  REDperiod=0  FEDperiod=0  REDperiod_sec=0  FEDperiod_sec=0  LoadModeDBRED=Immediate without using shadow  LoadModeDBFED=Immediate without using shadow  adcstartModuleA=off  adcrequestEventA=First event  adcstartEventA=Digital Compare Module A Event 1 start of conversion (DCAEVT1.soc)  adcstartEventA_type2=Counter equals to zero (CTR=Zero)  adcstartModuleB=off  adcrequestEventB=First event  adcstartEventB=Counter equals to zero (CTR=Zero)  adcstartEventB_type2=Counter equals to zero (CTR=Zero)  intEn=off  intPrd=First event  intSel=Counter equals to zero (CTR=Zero)  intSel_type2=Counter equals to zero (CTR=Zero)  hrpe=off  enHRPWM=off  HRPWM_LoadMode=Counter equals to period (CTR=PRD)  HRPWM_CTLMode=Duty or Period control mode  HRPWM_EDGMode=Both edge  hrpeb=off  enHRPWMB=off  HRPWM_LoadModeB=Counter equals to zero (CTR=ZERO)  HRPWM_CTLModeB=Duty or Period control mode  HRPWM_EDGModeB=Both edge  enHRDBRED=off  enHRDBFED=off  enSFO=on  enautoconv=on  chopperEnable=off  chopperFrequency=1  chopperFirstwidth=1  chopperDuty=12.5%  tripZonesource=Specify via dialog  tzselOSHT1=off  tzselOSHT2=off  tzselOSHT3=off  tzselOSHDCAEV1=off  tzselOSHDCBEV1=off  tzselCBC1=off  tzselCBC2=off  tzselCBC3=off  tzselCBCDCAEV2=off  tzselCBCDCBEV2=off  tzselOSHT4=off  tzselOSHT5=off  tzselOSHT6=off  tzselCBC4=off  tzselCBC5=off  tzselCBC6=off  enTzOstIntr=off  enTzCbcIntr=off  enTzDCAEVT1Intr=off  enTzDCAEVT2Intr=off  enTzDCBEVT1Intr=off  enTzDCBEVT2Intr=off  ePWMxAforced=No action  ePWMxBforced=No action  DCAEVT1forced=No action  DCBEVT1forced=No action  DCAEVT2forced=No action  DCBEVT2forced=No action  dcah=Trip Zone 1 input (TZ1)  dcal=Trip Zone 2 input (TZ2)  dcbh=Trip Zone 1 input (TZ1)  dcbl=Trip Zone 2 input (TZ2)  dcah_type2=GPTRIP1SEL/(TZ1)  dcal_type2=GPTRIP1SEL/(TZ1)  dcbh_type2=GPTRIP1SEL/(TZ1)  dcbl_type2=GPTRIP1SEL/(TZ1)  gendcaevt1=Event disabled  gendcaevt2=Event disabled  gendcbevt1=Event disabled  gendcbevt2=Event disabled  dcaevt1src=DCAEVT1 with sync  dcaevt2src=DCAEVT2 with sync  dcbevt1src=DCBEVT1 with sync  dcbevt2src=DCBEVT2 with sync  pulsesel=Counter equals to zero (CTR=Zero)  blankinv=off  blankoffset=0  blankwidth=0  evsrcsel=Filtered version of DCAEVT1 (DCAEVT1FILT)  encape=off
      settings: LibrarySourceBlock=c2837xDlib/ePWM
  ePWM7 : c2802xlib/ePWM  Commented=on  PwmType=C2000_Type4  useModule=ePWM6  ePWMxLINKTBPRD=Not Linked  periodUnits=Clock cycles  timerSource=Specify via dialog  timerPeriod_clk=4166  timerPeriod_sec=0.0001  tbshadow=Counter equals to zero  countingMode=Up-Down  phaseActiveEnable=Disable  phaseDirection=Count down after sync  phaseActive=0  synchronizationEnable=off  dcaevt1Sync=off  dcbevt1Sync=off  synchronizationOption=Disable  dcbevt1SyncOut=off  dcaevt1SyncOut=off  cmpdSyncOut=off  cmpcSyncOut=off  cmpbSyncOut=off  zeroSyncOut=off  swfSyncOut=off  perSynchronizationOption=Counter equals to period (CTR=PRD)  clockPrescale=1  HSclockPrescale=1  enswap=off  ePWMxAStatus=on  ePWMxAactionLogic1=Set  ePWMxAactionLogic2=Clear  ePWMxAactionLogic3=Clear  ePWMxAactionLogic4=Set  ePWMxAactionLogic5=Do nothing  ePWMxAactionLogic6=Do nothing  ePWMxACSFenable=off  ePWMxACSFvalue=Forcing disable  ePWMxASFreload=Zero  ePWMxBStatus=on  ePWMxBactionLogic1=Set  ePWMxBactionLogic2=Clear  ePWMxBactionLogic3=Do nothing  ePWMxBactionLogic4=Do nothing  ePWMxBactionLogic5=Clear  ePWMxBactionLogic6=Set  ePWMxBCSFenable=off  ePWMxBCSFvalue=Forcing disable  ePWMxBSFreload=Zero  ePWNxBOutWay=off  ePWMxLINKCMPA=Not Linked  CMPAUnits=Percentages  CMPASource=Input port  CMPAValue_per=50  CMPAValue_clk=32000  enCMPAshadow=Counter equals to zero (CTR=Zero)  ePWMxLINKCMPB=Not Linked  CMPBUnits=Percentages  CMPBSource=Input port  CMPBValue_per=50  CMPBValue_clk=32000  enCMPBshadow=Counter equals to zero (CTR=Zero)  ePWMxLINKCMPC=Not Linked  CMPCUnits=Clock cycles  CMPCSource=Specify via dialog  CMPCValue_per=50  CMPCValue_clk=32000  enCMPCshadow=Counter equals to zero (CTR=Zero)  ePWMxLINKCMPD=Not Linked  CMPDUnits=Clock cycles  CMPDSource=Specify via dialog  CMPDValue_per=50  CMPDValue_clk=32000  enCMPDshadow=Counter equals to zero (CTR=Zero)  enableDBePWMxA=off  enableDBePWMxB=off  enhalfcycle=off  DBpolarity=Active high (AH)  DBedgeDelay=Positive  DBSource_ePWMxA=ePWMxA  DBSource_ePWMxB=ePWMxA  DBPeriodUnits=Clock cycles  DBperiodSource=Specify via dialog  REDperiod=0  FEDperiod=0  REDperiod_sec=0  FEDperiod_sec=0  LoadModeDBRED=Immediate without using shadow  LoadModeDBFED=Immediate without using shadow  adcstartModuleA=off  adcrequestEventA=First event  adcstartEventA=Digital Compare Module A Event 1 start of conversion (DCAEVT1.soc)  adcstartEventA_type2=Counter equals to zero (CTR=Zero)  adcstartModuleB=off  adcrequestEventB=First event  adcstartEventB=Counter equals to zero (CTR=Zero)  adcstartEventB_type2=Counter equals to zero (CTR=Zero)  intEn=off  intPrd=First event  intSel=Counter equals to zero (CTR=Zero)  intSel_type2=Counter equals to zero (CTR=Zero)  hrpe=off  enHRPWM=off  HRPWM_LoadMode=Counter equals to period (CTR=PRD)  HRPWM_CTLMode=Duty or Period control mode  HRPWM_EDGMode=Both edge  hrpeb=off  enHRPWMB=off  HRPWM_LoadModeB=Counter equals to zero (CTR=ZERO)  HRPWM_CTLModeB=Duty or Period control mode  HRPWM_EDGModeB=Both edge  enHRDBRED=off  enHRDBFED=off  enSFO=on  enautoconv=on  chopperEnable=off  chopperFrequency=1  chopperFirstwidth=1  chopperDuty=12.5%  tripZonesource=Specify via dialog  tzselOSHT1=off  tzselOSHT2=off  tzselOSHT3=off  tzselOSHDCAEV1=off  tzselOSHDCBEV1=off  tzselCBC1=off  tzselCBC2=off  tzselCBC3=off  tzselCBCDCAEV2=off  tzselCBCDCBEV2=off  tzselOSHT4=off  tzselOSHT5=off  tzselOSHT6=off  tzselCBC4=off  tzselCBC5=off  tzselCBC6=off  enTzOstIntr=off  enTzCbcIntr=off  enTzDCAEVT1Intr=off  enTzDCAEVT2Intr=off  enTzDCBEVT1Intr=off  enTzDCBEVT2Intr=off  ePWMxAforced=No action  ePWMxBforced=No action  DCAEVT1forced=No action  DCBEVT1forced=No action  DCAEVT2forced=No action  DCBEVT2forced=No action  dcah=Trip Zone 1 input (TZ1)  dcal=Trip Zone 2 input (TZ2)  dcbh=Trip Zone 1 input (TZ1)  dcbl=Trip Zone 2 input (TZ2)  dcah_type2=GPTRIP1SEL/(TZ1)  dcal_type2=GPTRIP1SEL/(TZ1)  dcbh_type2=GPTRIP1SEL/(TZ1)  dcbl_type2=GPTRIP1SEL/(TZ1)  gendcaevt1=Event disabled  gendcaevt2=Event disabled  gendcbevt1=Event disabled  gendcbevt2=Event disabled  dcaevt1src=DCAEVT1 with sync  dcaevt2src=DCAEVT2 with sync  dcbevt1src=DCBEVT1 with sync  dcbevt2src=DCBEVT2 with sync  pulsesel=Counter equals to zero (CTR=Zero)  blankinv=off  blankoffset=0  blankwidth=0  evsrcsel=Filtered version of DCAEVT1 (DCAEVT1FILT)  encape=off
      settings: LibrarySourceBlock=c2837xDlib/ePWM
  ePWM8 : c2802xlib/ePWM  PwmType=C2000_Type4  useModule=ePWM8  ePWMxLINKTBPRD=Not Linked  periodUnits=Clock cycles  timerSource=Specify via dialog  timerPeriod_clk=4167  timerPeriod_sec=0.0001  tbshadow=Counter equals to zero  countingMode=Up-Down  phaseActiveEnable=Disable  phaseDirection=Count down after sync  phaseActive=0  synchronizationEnable=off  dcaevt1Sync=off  dcbevt1Sync=off  synchronizationOption=Disable  dcbevt1SyncOut=off  dcaevt1SyncOut=off  cmpdSyncOut=off  cmpcSyncOut=off  cmpbSyncOut=off  zeroSyncOut=off  swfSyncOut=off  perSynchronizationOption=Counter equals to period (CTR=PRD)  clockPrescale=1  HSclockPrescale=1  enswap=off  ePWMxAStatus=on  ePWMxAactionLogic1=Set  ePWMxAactionLogic2=Clear  ePWMxAactionLogic3=Clear  ePWMxAactionLogic4=Set  ePWMxAactionLogic5=Do nothing  ePWMxAactionLogic6=Do nothing  ePWMxACSFenable=off  ePWMxACSFvalue=Forcing disable  ePWMxASFreload=Zero  ePWMxBStatus=on  ePWMxBactionLogic1=Set  ePWMxBactionLogic2=Clear  ePWMxBactionLogic3=Do nothing  ePWMxBactionLogic4=Do nothing  ePWMxBactionLogic5=Clear  ePWMxBactionLogic6=Set  ePWMxBCSFenable=off  ePWMxBCSFvalue=Forcing disable  ePWMxBSFreload=Zero  ePWNxBOutWay=off  ePWMxLINKCMPA=Not Linked  CMPAUnits=Percentages  CMPASource=Input port  CMPAValue_per=50  CMPAValue_clk=32000  enCMPAshadow=Counter equals to zero (CTR=Zero)  ePWMxLINKCMPB=Not Linked  CMPBUnits=Percentages  CMPBSource=Input port  CMPBValue_per=50  CMPBValue_clk=32000  enCMPBshadow=Counter equals to zero (CTR=Zero)  ePWMxLINKCMPC=Not Linked  CMPCUnits=Clock cycles  CMPCSource=Specify via dialog  CMPCValue_per=50  CMPCValue_clk=32000  enCMPCshadow=Counter equals to zero (CTR=Zero)  ePWMxLINKCMPD=Not Linked  CMPDUnits=Clock cycles  CMPDSource=Specify via dialog  CMPDValue_per=50  CMPDValue_clk=32000  enCMPDshadow=Counter equals to zero (CTR=Zero)  enableDBePWMxA=off  enableDBePWMxB=off  enhalfcycle=off  DBpolarity=Active high (AH)  DBedgeDelay=Positive  DBSource_ePWMxA=ePWMxA  DBSource_ePWMxB=ePWMxA  DBPeriodUnits=Clock cycles  DBperiodSource=Specify via dialog  REDperiod=0  FEDperiod=0  REDperiod_sec=0  FEDperiod_sec=0  LoadModeDBRED=Immediate without using shadow  LoadModeDBFED=Immediate without using shadow  adcstartModuleA=off  adcrequestEventA=First event  adcstartEventA=Digital Compare Module A Event 1 start of conversion (DCAEVT1.soc)  adcstartEventA_type2=Counter equals to zero (CTR=Zero)  adcstartModuleB=off  adcrequestEventB=First event  adcstartEventB=Counter equals to zero (CTR=Zero)  adcstartEventB_type2=Counter equals to zero (CTR=Zero)  intEn=off  intPrd=First event  intSel=Counter equals to zero (CTR=Zero)  intSel_type2=Counter equals to zero (CTR=Zero)  hrpe=off  enHRPWM=off  HRPWM_LoadMode=Counter equals to period (CTR=PRD)  HRPWM_CTLMode=Duty or Period control mode  HRPWM_EDGMode=Both edge  hrpeb=off  enHRPWMB=off  HRPWM_LoadModeB=Counter equals to zero (CTR=ZERO)  HRPWM_CTLModeB=Duty or Period control mode  HRPWM_EDGModeB=Both edge  enHRDBRED=off  enHRDBFED=off  enSFO=on  enautoconv=on  chopperEnable=off  chopperFrequency=1  chopperFirstwidth=1  chopperDuty=12.5%  tripZonesource=Specify via dialog  tzselOSHT1=off  tzselOSHT2=off  tzselOSHT3=off  tzselOSHDCAEV1=off  tzselOSHDCBEV1=off  tzselCBC1=off  tzselCBC2=off  tzselCBC3=off  tzselCBCDCAEV2=off  tzselCBCDCBEV2=off  tzselOSHT4=off  tzselOSHT5=off  tzselOSHT6=off  tzselCBC4=off  tzselCBC5=off  tzselCBC6=off  enTzOstIntr=off  enTzCbcIntr=off  enTzDCAEVT1Intr=off  enTzDCAEVT2Intr=off  enTzDCBEVT1Intr=off  enTzDCBEVT2Intr=off  ePWMxAforced=No action  ePWMxBforced=No action  DCAEVT1forced=No action  DCBEVT1forced=No action  DCAEVT2forced=No action  DCBEVT2forced=No action  dcah=Trip Zone 1 input (TZ1)  dcal=Trip Zone 2 input (TZ2)  dcbh=Trip Zone 1 input (TZ1)  dcbl=Trip Zone 2 input (TZ2)  dcah_type2=GPTRIP1SEL/(TZ1)  dcal_type2=GPTRIP1SEL/(TZ1)  dcbh_type2=GPTRIP1SEL/(TZ1)  dcbl_type2=GPTRIP1SEL/(TZ1)  gendcaevt1=Event disabled  gendcaevt2=Event disabled  gendcbevt1=Event disabled  gendcbevt2=Event disabled  dcaevt1src=DCAEVT1 with sync  dcaevt2src=DCAEVT2 with sync  dcbevt1src=DCBEVT1 with sync  dcbevt2src=DCBEVT2 with sync  pulsesel=Counter equals to zero (CTR=Zero)  blankinv=off  blankoffset=0  blankwidth=0  evsrcsel=Filtered version of DCAEVT1 (DCAEVT1FILT)  encape=off
      settings: LibrarySourceBlock=c2837xDlib/ePWM
  iccp_DAB_adc : From  Commented=on  GotoTag=iccp_DAB_adc
  iccs_DAB_adc : From  Commented=on  GotoTag=iccs_DAB_adc
  pq Current : Subsystem
  wires:
  Constant15/1 -> ePWM2/2
  ADC4/1 -> Rate Transition12/1
  Gain26/1 -> Gain29/1
  Gain8/1 -> Add2/1
  Product9/1 -> ePWM20/1, Mux1/3
  Gain27/1 -> Gain28/1
  ADC6/1 -> Rate Transition14/1
  Gain17/1 -> Gain18/1
  Constant22/1 -> ePWM12/1
  Gain19/1 -> Gain22/1
  Gain9/1 -> Add5/1
  Constant19/1 -> Add5/2, Add2/2, Add1/2
  Gain12/1 -> Gain13/1
  Add5/1 -> Product9/2
  [m_c] -> Gain9/1
  [m_b] -> Gain8/1
  Gain24/1 -> Gain25/1
  Gain6/1 -> Add1/1
  [m_a] -> Gain6/1
  ADC12/1 -> Rate Transition4/1
  Gain5/1 -> Gain42/1
  Constant5/1 -> ePWM3/2
  ADC8/1 -> Rate Transition/1
  Gain/1 -> [ia_TNPC_pu]
  Gain3/1 -> Gain4/1
  Constant6/1 -> ePWM4/1
  Constant12/1 -> ePWM7/1
  Gain1/1 -> [ib_TNPC_pu]
  Porcent_D4/1 -> ePWM21/1, ePWM21/2, ePWM18/2, ePWM18/1, ePWM17/2, ePWM17/1
  Mux1/1 -> Scope6/1
  Constant24/1 -> ePWM13/1
  ADC11/1 -> Rate Transition3/1
  Gain4/1 -> Gain10/1
  Constant23/1 -> ePWM12/2
  Constant10/1 -> ePWM6/1
  ADC10/1 -> Rate Transition2/1
  Product7/1 -> ePWM19/1, Mux1/1
  ADC5/1 -> Rate Transition13/1
  ADC2/1 -> Rate Transition10/1
  Add1/1 -> Product7/2
  Gain2/1 -> Gain5/1
  Constant11/1 -> ePWM6/2
  Add2/1 -> Product8/2
  Constant25/1 -> ePWM13/2
  ADC1/1 -> Rate Transition9/1
  ADC3/1 -> Rate Transition11/1
  ADC/1 -> Rate Transition8/1
  Constant14/1 -> ePWM2/1
  [VccB_TNPC_adc] -> Gain33/1
  ADC15/1 -> Rate Transition7/1
  Constant3/1 -> ePWM1/2
  Data Store Read1/1 -> Gain7/1
  Data Store Read6/1 -> Digital Output2/1
  Gain7/1 -> Product7/1, Product8/1, Product9/1
  Constant9/1 -> ePWM5/2
  Gain32/1 -> Gain49/1
  ADC7/1 -> Rate Transition15/1
  Gain30/1 -> Gain31/1
  Constant8/1 -> ePWM5/1
  Constant1/1 -> ePWM1/1
  Gain14/1 -> Gain47/1
  Constant17/1 -> ePWM8/2
  iccp_DAB_adc/1 -> Gain14/1
  ADC14/1 -> Rate Transition6/1
  Gain34/1 -> Terminator5/1
  Gain33/1 -> Gain50/1
  Constant13/1 -> ePWM7/2
  Constant4/1 -> ePWM3/1
  ADC13/1 -> Rate Transition5/1
  [VccT_TNPC_adc] -> Gain32/1
  Product8/1 -> Mux1/2, ePWM22/1
  iccs_DAB_adc/1 -> Gain15/1
  Constant7/1 -> ePWM4/2
  Gain11/1 -> [ic_TNPC_pu]
  Gain13/1 -> Gain43/1
  Constant16/1 -> ePWM8/1
  ADC9/1 -> Rate Transition1/1
  Vcc_DAB_adc/1 -> Gain34/1
  Gain15/1 -> Gain48/1
  Gain20/1 -> Gain21/1
  [ia_TNPC_adc] -> Sum3/1
  Sum3/1 -> Gain3/1
  ADC_offset_ia_TNPC/1 -> Sum3/2
  [ib_TNPC_adc] -> Sum4/1
  Sum4/1 -> Gain2/1
  ADC_offset_ib_TNPC/1 -> Sum4/2
  ADC_offset_ic_TNPC/1 -> Sum5/2
  [ic_TNPC_adc] -> Sum5/1
  Sum5/1 -> Gain12/1
  [ia_GRID_adc] -> Sum6/1
  Sum6/1 -> Gain20/1
  ADC_offset_ia_GRID/1 -> Sum6/2
  [ib_GRID_adc] -> Sum7/1
  Sum7/1 -> Gain19/1
  ADC_offset_ib_GRID/1 -> Sum7/2
  [ic_GRID_adc] -> Sum8/1
  Sum8/1 -> Gain17/1
  ADC_offset_ic_GRID/1 -> Sum8/2
  Gain21/1 -> Gain44/1
  Gain22/1 -> Gain45/1
  Gain18/1 -> Gain46/1
  Sum9/1 -> Gain16/1
  Gain16/1 -> Gain23/1
  [Va_TNPC_adc] -> Sum9/1
  ADC_offset_va_TNPC/1 -> Sum9/2
  Gain28/1 -> Gain52/1
  [Vb_TNPC_adc] -> Sum10/1
  Sum10/1 -> Gain27/1
  ADC_offset_vb_TNPC/1 -> Sum10/2
  [Vc_TNPC_adc] -> Sum11/1
  Sum11/1 -> Gain26/1
  ADC_offset_vc_TNPC/1 -> Sum11/2
  Gain29/1 -> Gain53/1
  Gain25/1 -> Terminator21/1
  Vs_DAB_adc/1 -> Sum12/1
  Sum12/1 -> Gain24/1
  ADC_offset_vs_DAB/1 -> Sum12/2
  Vp_DAB_adc/1 -> Sum13/1
  Sum13/1 -> Gain30/1
  Gain31/1 -> Terminator4/1
  ADC_offset_vp_DAB/1 -> Sum13/2
  Gain39/1 -> [Va_TNPC_pu]
  Gain23/1 -> Gain51/1
  Gain40/1 -> [Vb_TNPC_pu]
  Gain41/1 -> [Vc_TNPC_pu]
  [ib_TNPC_pu] -> RMS_fcn1/1(RMSin)  "ib_TNPC_pu"
  [ia_TNPC_pu] -> RMS_fcn/1(RMSin)  "ia_TNPC_pu"
  [VccB_TNPC_pu] -> Sum2/2, Sum1/2
  Mux2/1 -> [i_TNPC_RMS]
  [ic_TNPC_pu] -> RMS_fcn2/1(RMSin)  "ic_TNPC_pu"
  Sum2/1 -> [Vunb_TNPC_pu]
  Sum1/1 -> [Vcc_TNPC_pu]  "Vdc_total"
  [VccT_TNPC_pu] -> Sum1/1, Sum2/1
  Rate Transition/1 -> Data Type Conversion/1
  Rate Transition1/1 -> Data Type Conversion1/1
  Rate Transition2/1 -> Data Type Conversion2/1
  Rate Transition3/1 -> Data Type Conversion3/1
  Rate Transition4/1 -> Data Type Conversion4/1
  Rate Transition5/1 -> Data Type Conversion5/1
  Rate Transition6/1 -> Data Type Conversion6/1
  Rate Transition7/1 -> Data Type Conversion7/1
  Rate Transition8/1 -> Data Type Conversion8/1
  Rate Transition9/1 -> Data Type Conversion9/1
  Rate Transition10/1 -> Data Type Conversion10/1
  Rate Transition11/1 -> Data Type Conversion11/1
  Rate Transition12/1 -> Data Type Conversion12/1
  Rate Transition13/1 -> Data Type Conversion13/1
  Rate Transition14/1 -> Data Type Conversion14/1
  Rate Transition15/1 -> Data Type Conversion15/1
  Data Type Conversion/1 -> [ia_TNPC_adc]
  Data Type Conversion1/1 -> [ib_TNPC_adc]
  Data Type Conversion2/1 -> [ic_TNPC_adc]
  Data Type Conversion3/1 -> [ib_GRID_adc]
  Data Type Conversion4/1 -> [ia_GRID_adc]
  Data Type Conversion5/1 -> [ic_GRID_adc]
  Data Type Conversion6/1 -> Goto10/1
  Data Type Conversion7/1 -> Goto11/1
  Data Type Conversion8/1 -> [Va_TNPC_adc]
  Data Type Conversion9/1 -> [Vb_TNPC_adc]
  Data Type Conversion10/1 -> [Vc_TNPC_adc]
  Data Type Conversion11/1 -> Goto15/1
  Data Type Conversion12/1 -> Goto16/1
  Data Type Conversion13/1 -> [VccT_TNPC_adc]
  Data Type Conversion14/1 -> [VccB_TNPC_adc]
  Data Type Conversion15/1 -> Goto19/1
  RMS_fcn/1(yout) -> Mux2/1  "ia_RMS_pu"
  RMS_fcn1/1(yout) -> Mux2/2  "ib_RMS_pu"
  RMS_fcn2/1(yout) -> Mux2/3  "ic_RMS_pu"
  [Va_TNPC_pu] -> RMS_fcn3/1(RMSin)
  [Vc_TNPC_pu] -> RMS_fcn5/1(RMSin)
  [Vb_TNPC_pu] -> RMS_fcn4/1(RMSin)
  RMS_fcn4/1(yout) -> Mux3/2  "Vb_RMS_pu"
  RMS_fcn3/1(yout) -> Mux3/1  "Va_RMS_pu"
  RMS_fcn5/1(yout) -> Mux3/3  "Vc_RMS_pu"
  Mux3/1 -> [V_TNPC_RMS]
  [OUT_GPIO] -> Digital Output3/1
  Data Store Read2/1 -> [enable], Digital Output1/1
  Compare To Constant/1 -> Digital Output4/1
  [ia_GRID_pu] -> Max/1  "ia_grid_pu"
  Max/1 -> Compare To Constant/1
  [ib_GRID_pu] -> Max/2  "ib_grid_pu"
  [ic_GRID_pu] -> Max/3  "ic_grid_pu"
  Gain65/1 -> [Q_ref_EV]
  Qref_SI/1 -> Gain65/1
  Gain64/1 -> [P_ref_EV]
  Gain63/1 -> Gain64/1
  Pref_SI/1 -> Saturation/1
  Saturation/1 -> Gain63/1
  MATLAB Function11/1(error_overcurrent) -> Data Store Write3/1
  [Vunb_TNPC_pu] -> MATLAB Function11/7(V_unb)
  MATLAB Function11/7(enable_PreCharge_out) -> Data Store Write7/1
  MATLAB Function11/9(enable_PQ_out) -> Data Store Write10/1
  Data Store Read5/1 -> MATLAB Function11/11(enable_PreCharge)
  Gain38/1 -> MATLAB Function11/8(Vunb_limit)
  [i_TNPC_RMS] -> MATLAB Function11/1(i_rms)
  Data Store Read3/1 -> MATLAB Function11/10(enable_PWM)
  Unbalance_Limit/1 -> Gain38/1
  MATLAB Function11/12(error_reset_out) -> Data Store Write/1
  Current_Limit/1 -> Gain35/1
  MATLAB Function11/4(error_unbalance) -> Data Store Write5/1
  MATLAB Function11/13(out_gpio) -> [OUT_GPIO]
  MATLAB Function11/5(error_low_Vdc) -> Data Store Write8/1
  MATLAB Function11/2(error_ac_overvoltage) -> Data Store Write6/1
  Data Store Read10/1 -> MATLAB Function11/13(enable_comp)
  MATLAB Function11/3(error_dc_overvoltage) -> Data Store Write4/1
  [Vcc_TNPC_pu] -> MATLAB Function11/5(V_dc)
  Gain37/1 -> MATLAB Function11/6(Vdc_limit)
  Gain36/1 -> MATLAB Function11/4(V_limit)
  MATLAB Function11/8(enable_PWM_out) -> Data Store Write1/1
  Data Store Read4/1 -> MATLAB Function11/9(enable_relay)
  MATLAB Function11/6(enable_contactor_out) -> Data Store Write2/1
  [V_TNPC_RMS] -> MATLAB Function11/3(V_rms)
  Gain35/1 -> MATLAB Function11/2(I_limit)
  AC_Voltage_Limit/1 -> Gain36/1
  Data Store Read9/1 -> MATLAB Function11/12(enable_PQ)
  Data Store Read/1 -> MATLAB Function11/14(error_reset)
  MATLAB Function11/11(enable_Feedforward_out) -> Data Store Write9/1
  DC_Voltage_Limit/1 -> Gain37/1
  MATLAB Function11/10(enable_comp_out) -> Data Store Write11/1
  Gain10/1 -> Gain/1
  Gain42/1 -> Gain1/1
  Gain43/1 -> Gain11/1
  Gain44/1 -> [ia_GRID_pu]
  Gain45/1 -> [ib_GRID_pu]
  Gain46/1 -> [ic_GRID_pu]
  Gain47/1 -> Terminator1/1
  Gain48/1 -> Terminator2/1
  Gain49/1 -> [VccT_TNPC_pu]
  Gain50/1 -> [VccB_TNPC_pu]
  Gain51/1 -> Gain39/1
  Gain52/1 -> Gain40/1
  Gain53/1 -> Gain41/1
  MATLAB Function3/1(alpha) -> [iGRID_alpha]  "i_GRID_alpha"
  [ib_TNPC_pu] -> MATLAB Function1/2(b)
  [Vgr_beta_unf] -> MATLAB Function4/1(v_unf)
  MATLAB Function5/2(beta) -> [il_beta]  "i_load_beta"
  MATLAB Function/1(v_f) -> [vPCC_alpha]  "v_PCC_alpha"
  [ib_load_pu] -> MATLAB Function5/2(b)
  MATLAB Function3/2(beta) -> [iGRID_beta]  "i_GRID_beta"
  [ia_load_pu] -> MATLAB Function5/1(a)
  [ic_load_pu] -> MATLAB Function5/3(c)
  [ib_GRID_pu] -> MATLAB Function3/2(b)
  MATLAB Function4/1(v_f) -> [vPCC_beta]  "v_PCC_beta"
  MATLAB Function1/1(alpha) -> [iTNPC_alpha]  "i_TNPC_alpha"
  Constant/1 -> MATLAB Function4/2(bD), MATLAB Function/2(bD)
  MATLAB Function2/1(alpha) -> [Vgr_alpha_unf]
  MATLAB Function1/2(beta) -> [iTNPC_beta]  "i_TNPC_beta"
  Constant20/1 -> MATLAB Function4/5(a2), MATLAB Function/5(a2)
  MATLAB Function2/2(beta) -> [Vgr_beta_unf]
  Constant2/1 -> MATLAB Function4/3(bQ), MATLAB Function/3(bQ)
  Sum/1 -> MATLAB Function2/3(c)
  [ic_TNPC_pu] -> MATLAB Function1/3(c)
  [ia_GRID_pu] -> MATLAB Function3/1(a)
  Constant18/1 -> MATLAB Function4/4(a1), MATLAB Function/4(a1)
  [ia_TNPC_pu] -> MATLAB Function1/1(a)
  [Va_TNPC_pu] -> MATLAB Function2/1(a), Sum/1
  Constant21/1 -> MATLAB Function4/6(enable), MATLAB Function/6(enable)
  [Vgr_alpha_unf] -> MATLAB Function/1(v_unf)
  MATLAB Function5/1(alpha) -> [il_alpha]  "i_load_alpha"
  [ic_GRID_pu] -> MATLAB Function3/3(c)
  [vPCC_beta] -> VoltVAr/2(v_beta)
  [enable_comp] -> VoltVAr/3(enable)
  Current Controller/3(mc) -> [m_c]  "mod_c"
  [vPCC_beta] -> pq Current/4(V_beta)
  [vPCC_beta] -> Compensation Reference/4(v_beta)
  Constant27/1 -> PQref Calculation/8(q_VoltVAr)
  pq Current/2(i_beta) -> [i_beta_ref]
  Data Store Read7/1 -> [enable_comp]
  [P_ref] -> pq Current/1(p)
  [enable_pq] -> PQref Calculation/11(enable_pq)
  Current Controller/2(mb) -> [m_b]  "mod_b"
  [P_ref_EV] -> PQref Calculation/1(p_EV)
  VoltVAr/2(q_VoltVAr) -> Terminator/1
  [iTNPC_beta] -> Current Controller/4(i_beta)
  [vPCC_alpha] -> VoltVAr/1(v_alpha)
  [V_rms] -> PQref Calculation/9(Voltage)
  [enable] -> Current Controller/7(enable)
  Compensation Reference/1(p_avg) -> [p_avg_comp]
  Compensation Reference/4(q_osc) -> [q_osc_comp]
  [q_osc_comp] -> PQref Calculation/7(q_osc_comp)
  Compensation Reference/3(q_avg) -> [q_avg_comp]
  [il_alpha] -> Compensation Reference/1(i_alpha)
  [enable_pq] -> Compensation Reference/6(enable_pq)
  [P_ref_EV] -> Compensation Reference/5(p_EV)
  [vPCC_alpha] -> Compensation Reference/3(v_alpha)
  VoltVAr/1(V_rms) -> [V_rms]  "V_RMS"
  Compensation Reference/2(p_osc) -> [p_osc_comp]
  [iTNPC_alpha] -> Current Controller/2(i_alpha)
  [vPCC_alpha] -> Current Controller/5(v_alpha)  "Va_inPLL"
  [THDi_load] -> PQref Calculation/10(THDi)
  [i_beta_ref] -> Current Controller/3(iref_beta)  "iref_beta"
  Constant26/1 -> PQref Calculation/3(p_Vdc)
  Compensation Reference/5(THDi) -> [THDi_load]
  [p_avg_comp] -> PQref Calculation/4(p_avg_comp)
  PQref Calculation/1(P_ref) -> [P_ref]  "P_ref"
  [enable_comp] -> PQref Calculation/12(enable_comp)
  [il_beta] -> Compensation Reference/2(i_beta)
  [vPCC_alpha] -> pq Current/3(V_alpha)
  pq Current/1(i_alpha) -> [i_alpha_ref]
  Data Store Read8/1 -> [enable_pq]
  PQref Calculation/2(Q_ref) -> [Q_ref]  "Q_ref"
  [i_alpha_ref] -> Current Controller/1(iref_alpha)  "iref_alpha"
  [Q_ref] -> pq Current/2(q)
  [Q_ref_EV] -> PQref Calculation/2(q_EV)
  [vPCC_beta] -> Current Controller/6(v_beta)
  [p_osc_comp] -> PQref Calculation/5(p_osc_comp)
  [enable_pq] -> pq Current/5(Enable2)
  Current Controller/1(ma) -> [m_a]  "mod_a"
  [q_avg_comp] -> PQref Calculation/6(q_avg_comp)
  [ib_TNPC_pu] -> Sum15/1
  Gain56/1 -> [ic_load_pu]
  [ic_TNPC_pu] -> Sum16/1
  Gain54/1 -> [ia_load_pu]
  Sum16/1 -> Gain56/1
  [ib_GRID_pu] -> Sum15/2
  [ic_GRID_pu] -> Sum16/2
  Sum15/1 -> Gain55/1
  [ia_GRID_pu] -> Sum14/2
  Gain55/1 -> [ib_load_pu]
  [ia_TNPC_pu] -> Sum14/1
  Sum14/1 -> Gain54/1
  [lPF_GR] -> Scope17/2  "PF"
  MATLAB Function6/1(p_avg) -> Terminator11/1  "pA_L"
  MATLAB Function6/4(q_osc) -> Terminator8/1  "qO_L"
  [vPCC_beta] -> MATLAB Function8/4(v_beta)
  Gain57/1 -> Scope17/3  "THD"
  MATLAB Function9/2(lambda_PF) -> [lPF_GR]
  [il_alpha] -> MATLAB Function6/1(i_alpha)
  [V_rms] -> Scope17/4  "V_rms"
  [vPCC_beta] -> MATLAB Function9/4(v_beta)
  [iGRID_alpha] -> MATLAB Function9/1(i_alpha)
  [THD_GR] -> Gain57/1
  MATLAB Function8/4(q_osc) -> Terminator12/1  "qO_EV"
  [qa_GR] -> MATLAB Function9/6(q_avg)
  [pa_GR] -> MATLAB Function9/5(p_avg)
  [vPCC_beta] -> MATLAB Function6/4(v_beta)
  [iGRID_beta] -> MATLAB Function7/2(i_beta)
  MATLAB Function7/2(p_osc) -> Terminator6/1  "pO_GR"
  MATLAB Function9/3(THDi) -> [THD_GR]
  MATLAB Function9/1(lambda_Q) -> [lQ_GR]
  [vPCC_alpha] -> MATLAB Function6/3(v_alpha)
  [iGRID_beta] -> MATLAB Function9/2(i_beta)
  MATLAB Function7/1(p_avg) -> [pa_GR]  "pA_GR"
  [iTNPC_beta] -> MATLAB Function8/2(i_beta)
  [iTNPC_alpha] -> MATLAB Function8/1(i_alpha)
  [iGRID_alpha] -> MATLAB Function7/1(i_alpha)
  MATLAB Function9/4(S_fund) -> Terminator3/1
  MATLAB Function8/3(q_avg) -> Terminator13/1  "qA_EV"
  [lQ_GR] -> Scope17/1  "PF_Q"
  [vPCC_beta] -> MATLAB Function7/4(v_beta)
  MATLAB Function8/2(p_osc) -> Terminator14/1  "pO_EV"
  MATLAB Function6/2(p_osc) -> Terminator10/1  "pO_L"
  MATLAB Function7/3(q_avg) -> [qa_GR]  "qA_GR"
  [vPCC_alpha] -> MATLAB Function9/3(v_alpha)
  MATLAB Function7/4(q_osc) -> Terminator7/1  "qO_GR"
  MATLAB Function8/1(p_avg) -> Terminator15/1  "pA_EV"
  [vPCC_alpha] -> MATLAB Function8/3(v_alpha)
  [il_beta] -> MATLAB Function6/2(i_beta)
  [vPCC_alpha] -> MATLAB Function7/3(v_alpha)
  MATLAB Function6/3(q_avg) -> Terminator9/1  "qA_L"
  [Vb_TNPC_pu] -> Sum/2, MATLAB Function2/2(b)
